simulink model "ADCS_v1"  (R2026a)
settings: Solver=VariableStepAuto  StopTime=t0  FixedStep=0.1  MaxStep=0.1
model workspace (MAT data in the model file):
  i = 8
  omega_thr = 1
  simIn = Simulink.SimulationInput
  simIn.ExternalInput = Simulink.SimulationData.Dataset
  simIn.ExternalInput.any.Name = ''
  simIn.ExternalInput.any.Version = 3
  simIn.ExternalInput.any.Storage = Simulink.SimulationData.Storage.RamDatasetStorage
  simIn.ExternalInput.any.Storage.any.Version = 2
  simIn.ExternalInput.any.Storage.any.Elements{1} = timeseries
  simIn.ExternalInput.any.Storage.any.Elements{1}.Name = 'u1'
  simIn.ExternalInput.any.Storage.any.Elements{1}.DataInfo = tsdata.datametadata
  simIn.ExternalInput.any.Storage.any.Elements{1}.DataInfo.Interpolation = tsdata.interpolation
  simIn.ExternalInput.any.Storage.any.Elements{1}.DataInfo.Interpolation.Fhandle : function handle (value not decoded)
  simIn.ExternalInput.any.Storage.any.Elements{1}.DataInfo.Interpolation.Name = 'linear'
  simIn.ExternalInput.any.Storage.any.Elements{1}.TimeInfo = tsdata.timemetadata
  simIn.ExternalInput.any.Storage.any.Elements{1}.TimeInfo.Length = 101
  simIn.ExternalInput.any.Storage.any.Elements{1}.TimeInfo.DuplicateTimes = 0
  simIn.ExternalInput.any.Storage.any.Elements{1}.TimeInfo.Time_ = [0; 0.1; 0.2; 0.3; 0.4; 0.5; 0.6; 0.7; 0.8; 0.9; 1; 1.1; 1.2; 1.3; 1.4; 1.5; 1.6; 1.7; 1.8; 1.9; 2; 2.1; 2.2; 2.3; 2.4; 2.5; 2.6; 2.7; 2.8; 2.9; 3; 3.1; 3.2; 3.3; 3.4; 3.5; 3.6; 3.7; 3.8; 3.9; 4; 4.1; 4.2; 4.3; 4.4; 4.5; 4.6; 4.7; 4.8; 4.9; 5; 5.1; 5.2; 5.3; 5.4; 5.5; 5.6; 5.7; 5.8; 5.9; 6; 6.1; 6.2; 6.3; 6.4; 6.5; 6.6; 6.7; 6.8; 6.9; 7; 7.1; 7.2; 7.3; 7.4; 7.5; 7.6; 7.7; 7.8; 7.9; 8; 8.1; 8.2; 8.3; 8.4; 8.5; 8.6; 8.7; 8.8; 8.9; 9; 9.1; 9.2; 9.3; 9.4; 9.5; 9.6; 9.7; 9.8; 9.9; 10]
  simIn.ExternalInput.any.Storage.any.Elements{1}.TimeInfo.Initialized = 1
  simIn.ExternalInput.any.Storage.any.Elements{1}.QualityInfo = tsdata.qualmetadata
  simIn.ExternalInput.any.Storage.any.Elements{1}.Data_ = [12; 12; 12; 12; 12; 12; 12; 12; 12; 12; 12; 12; 12; 12; 12; 12; 12; 12; 12; 12; 12; 12; 12; 12; 12; 12; 12; 12; 12; 12; 12; 12; 12; 12; 12; 12; 12; 12; 12; 12; 12; 12; 12; 12; 12; 12; 12; 12; 12; 12; 12; 12; 12; 12; 12; 12; 12; 12; 12; 12; 12; 12; 12; 12; 12; 12; 12; 12; 12; 12; 12; 12; 12; 12; 12; 12; 12; 12; 12; 12; 12; 12; 12; 12; 12; 12; 12; 12; 12; 12; 12; 12; 12; 12; 12; 12; 12; 12; 12; 12; 12]
  simIn.ExternalInput.any.Storage.any.Elements{2} = timeseries
  simIn.ExternalInput.any.Storage.any.Elements{2}.Name = 'u2'
  simIn.ExternalInput.any.Storage.any.Elements{2}.DataInfo = tsdata.datametadata
  simIn.ExternalInput.any.Storage.any.Elements{2}.DataInfo.Interpolation = tsdata.interpolation
  simIn.ExternalInput.any.Storage.any.Elements{2}.DataInfo.Interpolation.Fhandle : function handle (value not decoded)
  simIn.ExternalInput.any.Storage.any.Elements{2}.DataInfo.Interpolation.Name = 'linear'
  simIn.ExternalInput.any.Storage.any.Elements{2}.TimeInfo = tsdata.timemetadata
  simIn.ExternalInput.any.Storage.any.Elements{2}.TimeInfo.Length = 101
  simIn.ExternalInput.any.Storage.any.Elements{2}.TimeInfo.DuplicateTimes = 0
  simIn.ExternalInput.any.Storage.any.Elements{2}.TimeInfo.Time_ = [0; 0.1; 0.2; 0.3; 0.4; 0.5; 0.6; 0.7; 0.8; 0.9; 1; 1.1; 1.2; 1.3; 1.4; 1.5; 1.6; 1.7; 1.8; 1.9; 2; 2.1; 2.2; 2.3; 2.4; 2.5; 2.6; 2.7; 2.8; 2.9; 3; 3.1; 3.2; 3.3; 3.4; 3.5; 3.6; 3.7; 3.8; 3.9; 4; 4.1; 4.2; 4.3; 4.4; 4.5; 4.6; 4.7; 4.8; 4.9; 5; 5.1; 5.2; 5.3; 5.4; 5.5; 5.6; 5.7; 5.8; 5.9; 6; 6.1; 6.2; 6.3; 6.4; 6.5; 6.6; 6.7; 6.8; 6.9; 7; 7.1; 7.2; 7.3; 7.4; 7.5; 7.6; 7.7; 7.8; 7.9; 8; 8.1; 8.2; 8.3; 8.4; 8.5; 8.6; 8.7; 8.8; 8.9; 9; 9.1; 9.2; 9.3; 9.4; 9.5; 9.6; 9.7; 9.8; 9.9; 10]
  simIn.ExternalInput.any.Storage.any.Elements{2}.TimeInfo.Initialized = 1
  simIn.ExternalInput.any.Storage.any.Elements{2}.QualityInfo = tsdata.qualmetadata
  simIn.ExternalInput.any.Storage.any.Elements{2}.Data_ = [1; 1; 1; 1; 1; 1; 1; 1; 1; 1; 1; 1; 1; 1; 1; 1; 1; 1; 1; 1; 1; 1; 1; 1; 1; 1; 1; 1; 1; 1; 1; 1; 1; 1; 1; 1; 1; 1; 1; 1; 1; 1; 1; 1; 1; 1; 1; 1; 1; 1; 1; 1; 1; 1; 1; 1; 1; 1; 1; 1; 1; 1; 1; 1; 1; 1; 1; 1; 1; 1; 1; 1; 1; 1; 1; 1; 1; 1; 1; 1; 1; 1; 1; 1; 1; 1; 1; 1; 1; 1; 1; 1; 1; 1; 1; 1; 1; 1; 1; 1; 1]
  simIn.ExternalInput.any.Storage.any.Elements{3} = timeseries
  simIn.ExternalInput.any.Storage.any.Elements{3}.Name = 'u3'
  simIn.ExternalInput.any.Storage.any.Elements{3}.DataInfo = tsdata.datametadata
  simIn.ExternalInput.any.Storage.any.Elements{3}.DataInfo.Interpolation = tsdata.interpolation
  simIn.ExternalInput.any.Storage.any.Elements{3}.DataInfo.Interpolation.Fhandle : function handle (value not decoded)
  simIn.ExternalInput.any.Storage.any.Elements{3}.DataInfo.Interpolation.Name = 'linear'
  simIn.ExternalInput.any.Storage.any.Elements{3}.TimeInfo = tsdata.timemetadata
  simIn.ExternalInput.any.Storage.any.Elements{3}.TimeInfo.Length = 101
  simIn.ExternalInput.any.Storage.any.Elements{3}.TimeInfo.DuplicateTimes = 0
  simIn.ExternalInput.any.Storage.any.Elements{3}.TimeInfo.Time_ = [0; 0.1; 0.2; 0.3; 0.4; 0.5; 0.6; 0.7; 0.8; 0.9; 1; 1.1; 1.2; 1.3; 1.4; 1.5; 1.6; 1.7; 1.8; 1.9; 2; 2.1; 2.2; 2.3; 2.4; 2.5; 2.6; 2.7; 2.8; 2.9; 3; 3.1; 3.2; 3.3; 3.4; 3.5; 3.6; 3.7; 3.8; 3.9; 4; 4.1; 4.2; 4.3; 4.4; 4.5; 4.6; 4.7; 4.8; 4.9; 5; 5.1; 5.2; 5.3; 5.4; 5.5; 5.6; 5.7; 5.8; 5.9; 6; 6.1; 6.2; 6.3; 6.4; 6.5; 6.6; 6.7; 6.8; 6.9; 7; 7.1; 7.2; 7.3; 7.4; 7.5; 7.6; 7.7; 7.8; 7.9; 8; 8.1; 8.2; 8.3; 8.4; 8.5; 8.6; 8.7; 8.8; 8.9; 9; 9.1; 9.2; 9.3; 9.4; 9.5; 9.6; 9.7; 9.8; 9.9; 10]
  simIn.ExternalInput.any.Storage.any.Elements{3}.TimeInfo.Initialized = 1
  simIn.ExternalInput.any.Storage.any.Elements{3}.QualityInfo = tsdata.qualmetadata
  simIn.ExternalInput.any.Storage.any.Elements{3}.Data_ = [0; 0; 0; 0; 0; 0; 0; 0; 0; 0; 0; 0; 0; 0; 0; 0; 0; 0; 0; 0; 0; 0; 0; 0; 0; 0; 0; 0; 0; 0; 0; 0; 0; 0; 0; 0; 0; 0; 0; 0; 0; 0; 0; 0; 0; 0; 0; 0; 0; 0; 0; 0; 0; 0; 0; 0; 0; 0; 0; 0; 0; 0; 0; 0; 0; 0; 0; 0; 0; 0; 0; 0; 0; 0; 0; 0; 0; 0; 0; 0; 0; 0; 0; 0; 0; 0; 0; 0; 0; 0; 0; 0; 0; 0; 0; 0; 0; 0; 0; 0; 0]
  simIn.ExternalInput.any.Storage.any.Elements{4} = timeseries
  simIn.ExternalInput.any.Storage.any.Elements{4}.Name = 'u4'
  simIn.ExternalInput.any.Storage.any.Elements{4}.DataInfo = tsdata.datametadata
  simIn.ExternalInput.any.Storage.any.Elements{4}.DataInfo.Interpolation = tsdata.interpolation
  simIn.ExternalInput.any.Storage.any.Elements{4}.DataInfo.Interpolation.Fhandle : function handle (value not decoded)
  simIn.ExternalInput.any.Storage.any.Elements{4}.DataInfo.Interpolation.Name = 'linear'
  simIn.ExternalInput.any.Storage.any.Elements{4}.TimeInfo = tsdata.timemetadata
  simIn.ExternalInput.any.Storage.any.Elements{4}.TimeInfo.Length = 101
  simIn.ExternalInput.any.Storage.any.Elements{4}.TimeInfo.DuplicateTimes = 0
  simIn.ExternalInput.any.Storage.any.Elements{4}.TimeInfo.Time_ = [0; 0.1; 0.2; 0.3; 0.4; 0.5; 0.6; 0.7; 0.8; 0.9; 1; 1.1; 1.2; 1.3; 1.4; 1.5; 1.6; 1.7; 1.8; 1.9; 2; 2.1; 2.2; 2.3; 2.4; 2.5; 2.6; 2.7; 2.8; 2.9; 3; 3.1; 3.2; 3.3; 3.4; 3.5; 3.6; 3.7; 3.8; 3.9; 4; 4.1; 4.2; 4.3; 4.4; 4.5; 4.6; 4.7; 4.8; 4.9; 5; 5.1; 5.2; 5.3; 5.4; 5.5; 5.6; 5.7; 5.8; 5.9; 6; 6.1; 6.2; 6.3; 6.4; 6.5; 6.6; 6.7; 6.8; 6.9; 7; 7.1; 7.2; 7.3; 7.4; 7.5; 7.6; 7.7; 7.8; 7.9; 8; 8.1; 8.2; 8.3; 8.4; 8.5; 8.6; 8.7; 8.8; 8.9; 9; 9.1; 9.2; 9.3; 9.4; 9.5; 9.6; 9.7; 9.8; 9.9; 10]
  simIn.ExternalInput.any.Storage.any.Elements{4}.TimeInfo.Initialized = 1
  simIn.ExternalInput.any.Storage.any.Elements{4}.QualityInfo = tsdata.qualmetadata
  simIn.ExternalInput.any.Storage.any.Elements{4}.Data_ = [1; 1; 1; 1; 1; 1; 1; 1; 1; 1; 1; 1; 1; 1; 1; 1; 1; 1; 1; 1; 1; 1; 1; 1; 1; 1; 1; 1; 1; 1; 1; 1; 1; 1; 1; 1; 1; 1; 1; 1; 1; 1; 1; 1; 1; 1; 1; 1; 1; 1; 1; 1; 1; 1; 1; 1; 1; 1; 1; 1; 1; 1; 1; 1; 1; 1; 1; 1; 1; 1; 1; 1; 1; 1; 1; 1; 1; 1; 1; 1; 1; 1; 1; 1; 1; 1; 1; 1; 1; 1; 1; 1; 1; 1; 1; 1; 1; 1; 1; 1; 1]
  simIn.ExternalInput.any.Storage.any.Elements{5} = timeseries
  simIn.ExternalInput.any.Storage.any.Elements{5}.Name = 'u5'
  simIn.ExternalInput.any.Storage.any.Elements{5}.DataInfo = tsdata.datametadata
  simIn.ExternalInput.any.Storage.any.Elements{5}.DataInfo.Interpolation = tsdata.interpolation
  simIn.ExternalInput.any.Storage.any.Elements{5}.DataInfo.Interpolation.Fhandle : function handle (value not decoded)
  simIn.ExternalInput.any.Storage.any.Elements{5}.DataInfo.Interpolation.Name = 'linear'
  simIn.ExternalInput.any.Storage.any.Elements{5}.TimeInfo = tsdata.timemetadata
  simIn.ExternalInput.any.Storage.any.Elements{5}.TimeInfo.Length = 101
  simIn.ExternalInput.any.Storage.any.Elements{5}.TimeInfo.DuplicateTimes = 0
  simIn.ExternalInput.any.Storage.any.Elements{5}.TimeInfo.Time_ = [0; 0.1; 0.2; 0.3; 0.4; 0.5; 0.6; 0.7; 0.8; 0.9; 1; 1.1; 1.2; 1.3; 1.4; 1.5; 1.6; 1.7; 1.8; 1.9; 2; 2.1; 2.2; 2.3; 2.4; 2.5; 2.6; 2.7; 2.8; 2.9; 3; 3.1; 3.2; 3.3; 3.4; 3.5; 3.6; 3.7; 3.8; 3.9; 4; 4.1; 4.2; 4.3; 4.4; 4.5; 4.6; 4.7; 4.8; 4.9; 5; 5.1; 5.2; 5.3; 5.4; 5.5; 5.6; 5.7; 5.8; 5.9; 6; 6.1; 6.2; 6.3; 6.4; 6.5; 6.6; 6.7; 6.8; 6.9; 7; 7.1; 7.2; 7.3; 7.4; 7.5; 7.6; 7.7; 7.8; 7.9; 8; 8.1; 8.2; 8.3; 8.4; 8.5; 8.6; 8.7; 8.8; 8.9; 9; 9.1; 9.2; 9.3; 9.4; 9.5; 9.6; 9.7; 9.8; 9.9; 10]
  simIn.ExternalInput.any.Storage.any.Elements{5}.TimeInfo.Initialized = 1
  simIn.ExternalInput.any.Storage.any.Elements{5}.QualityInfo = tsdata.qualmetadata
  simIn.ExternalInput.any.Storage.any.Elements{5}.Data_ = [0; 0; 0; 0; 0; 0; 0; 0; 0; 0; 0; 0; 0; 0; 0; 0; 0; 0; 0; 0; 0; 0; 0; 0; 0; 0; 0; 0; 0; 0; 0; 0; 0; 0; 0; 0; 0; 0; 0; 0; 0; 0; 0; 0; 0; 0; 0; 0; 0; 0; 0; 0; 0; 0; 0; 0; 0; 0; 0; 0; 0; 0; 0; 0; 0; 0; 0; 0; 0; 0; 0; 0; 0; 0; 0; 0; 0; 0; 0; 0; 0; 0; 0; 0; 0; 0; 0; 0; 0; 0; 0; 0; 0; 0; 0; 0; 0; 0; 0; 0; 0]
  simIn.ExternalInput.any.Storage.any.Elements{6} = timeseries
  simIn.ExternalInput.any.Storage.any.Elements{6}.Name = 'u6'
  simIn.ExternalInput.any.Storage.any.Elements{6}.DataInfo = tsdata.datametadata
  simIn.ExternalInput.any.Storage.any.Elements{6}.DataInfo.Interpolation = tsdata.interpolation
  simIn.ExternalInput.any.Storage.any.Elements{6}.DataInfo.Interpolation.Fhandle : function handle (value not decoded)
  simIn.ExternalInput.any.Storage.any.Elements{6}.DataInfo.Interpolation.Name = 'linear'
  simIn.ExternalInput.any.Storage.any.Elements{6}.TimeInfo = tsdata.timemetadata
  simIn.ExternalInput.any.Storage.any.Elements{6}.TimeInfo.Length = 101
  simIn.ExternalInput.any.Storage.any.Elements{6}.TimeInfo.DuplicateTimes = 0
  simIn.ExternalInput.any.Storage.any.Elements{6}.TimeInfo.Time_ = [0; 0.1; 0.2; 0.3; 0.4; 0.5; 0.6; 0.7; 0.8; 0.9; 1; 1.1; 1.2; 1.3; 1.4; 1.5; 1.6; 1.7; 1.8; 1.9; 2; 2.1; 2.2; 2.3; 2.4; 2.5; 2.6; 2.7; 2.8; 2.9; 3; 3.1; 3.2; 3.3; 3.4; 3.5; 3.6; 3.7; 3.8; 3.9; 4; 4.1; 4.2; 4.3; 4.4; 4.5; 4.6; 4.7; 4.8; 4.9; 5; 5.1; 5.2; 5.3; 5.4; 5.5; 5.6; 5.7; 5.8; 5.9; 6; 6.1; 6.2; 6.3; 6.4; 6.5; 6.6; 6.7; 6.8; 6.9; 7; 7.1; 7.2; 7.3; 7.4; 7.5; 7.6; 7.7; 7.8; 7.9; 8; 8.1; 8.2; 8.3; 8.4; 8.5; 8.6; 8.7; 8.8; 8.9; 9; 9.1; 9.2; 9.3; 9.4; 9.5; 9.6; 9.7; 9.8; 9.9; 10]
  simIn.ExternalInput.any.Storage.any.Elements{6}.TimeInfo.Initialized = 1
  simIn.ExternalInput.any.Storage.any.Elements{6}.QualityInfo = tsdata.qualmetadata
  simIn.ExternalInput.any.Storage.any.Elements{6}.Data_ = [1; 1; 1; 1; 1; 1; 1; 1; 1; 1; 1; 1; 1; 1; 1; 1; 1; 1; 1; 1; 1; 1; 1; 1; 1; 1; 1; 1; 1; 1; 1; 1; 1; 1; 1; 1; 1; 1; 1; 1; 1; 1; 1; 1; 1; 1; 1; 1; 1; 1; 1; 1; 1; 1; 1; 1; 1; 1; 1; 1; 1; 1; 1; 1; 1; 1; 1; 1; 1; 1; 1; 1; 1; 1; 1; 1; 1; 1; 1; 1; 1; 1; 1; 1; 1; 1; 1; 1; 1; 1; 1; 1; 1; 1; 1; 1; 1; 1; 1; 1; 1]
  simIn.ExternalInput.any.Storage.any.Elements{7} = timeseries
  simIn.ExternalInput.any.Storage.any.Elements{7}.Name = 'u7'
  simIn.ExternalInput.any.Storage.any.Elements{7}.DataInfo = tsdata.datametadata
  simIn.ExternalInput.any.Storage.any.Elements{7}.DataInfo.Interpolation = tsdata.interpolation
  simIn.ExternalInput.any.Storage.any.Elements{7}.DataInfo.Interpolation.Fhandle : function handle (value not decoded)
  simIn.ExternalInput.any.Storage.any.Elements{7}.DataInfo.Interpolation.Name = 'linear'
  simIn.ExternalInput.any.Storage.any.Elements{7}.TimeInfo = tsdata.timemetadata
  simIn.ExternalInput.any.Storage.any.Elements{7}.TimeInfo.Length = 101
  simIn.ExternalInput.any.Storage.any.Elements{7}.TimeInfo.DuplicateTimes = 0
  simIn.ExternalInput.any.Storage.any.Elements{7}.TimeInfo.Time_ = [0; 0.1; 0.2; 0.3; 0.4; 0.5; 0.6; 0.7; 0.8; 0.9; 1; 1.1; 1.2; 1.3; 1.4; 1.5; 1.6; 1.7; 1.8; 1.9; 2; 2.1; 2.2; 2.3; 2.4; 2.5; 2.6; 2.7; 2.8; 2.9; 3; 3.1; 3.2; 3.3; 3.4; 3.5; 3.6; 3.7; 3.8; 3.9; 4; 4.1; 4.2; 4.3; 4.4; 4.5; 4.6; 4.7; 4.8; 4.9; 5; 5.1; 5.2; 5.3; 5.4; 5.5; 5.6; 5.7; 5.8; 5.9; 6; 6.1; 6.2; 6.3; 6.4; 6.5; 6.6; 6.7; 6.8; 6.9; 7; 7.1; 7.2; 7.3; 7.4; 7.5; 7.6; 7.7; 7.8; 7.9; 8; 8.1; 8.2; 8.3; 8.4; 8.5; 8.6; 8.7; 8.8; 8.9; 9; 9.1; 9.2; 9.3; 9.4; 9.5; 9.6; 9.7; 9.8; 9.9; 10]
  simIn.ExternalInput.any.Storage.any.Elements{7}.TimeInfo.Initialized = 1
  simIn.ExternalInput.any.Storage.any.Elements{7}.QualityInfo = tsdata.qualmetadata
  simIn.ExternalInput.any.Storage.any.Elements{7}.Data_ = [1; 1; 1; 1; 1; 1; 1; 1; 1; 1; 1; 1; 1; 1; 1; 1; 1; 1; 1; 1; 1; 1; 1; 1; 1; 1; 1; 1; 1; 1; 1; 1; 1; 1; 1; 1; 1; 1; 1; 1; 1; 1; 1; 1; 1; 1; 1; 1; 1; 1; 1; 1; 1; 1; 1; 1; 1; 1; 1; 1; 1; 1; 1; 1; 1; 1; 1; 1; 1; 1; 1; 1; 1; 1; 1; 1; 1; 1; 1; 1; 1; 1; 1; 1; 1; 1; 1; 1; 1; 1; 1; 1; 1; 1; 1; 1; 1; 1; 1; 1; 1]
  simIn.ExternalInput.any.Storage.any.Elements{8} = timeseries
  simIn.ExternalInput.any.Storage.any.Elements{8}.Name = 'u8'
  simIn.ExternalInput.any.Storage.any.Elements{8}.DataInfo = tsdata.datametadata
  simIn.ExternalInput.any.Storage.any.Elements{8}.DataInfo.Interpolation = tsdata.interpolation
  simIn.ExternalInput.any.Storage.any.Elements{8}.DataInfo.Interpolation.Fhandle : function handle (value not decoded)
  simIn.ExternalInput.any.Storage.any.Elements{8}.DataInfo.Interpolation.Name = 'linear'
  simIn.ExternalInput.any.Storage.any.Elements{8}.TimeInfo = tsdata.timemetadata
  simIn.ExternalInput.any.Storage.any.Elements{8}.TimeInfo.Length = 101
  simIn.ExternalInput.any.Storage.any.Elements{8}.TimeInfo.DuplicateTimes = 0
  simIn.ExternalInput.any.Storage.any.Elements{8}.TimeInfo.Time_ = [0; 0.1; 0.2; 0.3; 0.4; 0.5; 0.6; 0.7; 0.8; 0.9; 1; 1.1; 1.2; 1.3; 1.4; 1.5; 1.6; 1.7; 1.8; 1.9; 2; 2.1; 2.2; 2.3; 2.4; 2.5; 2.6; 2.7; 2.8; 2.9; 3; 3.1; 3.2; 3.3; 3.4; 3.5; 3.6; 3.7; 3.8; 3.9; 4; 4.1; 4.2; 4.3; 4.4; 4.5; 4.6; 4.7; 4.8; 4.9; 5; 5.1; 5.2; 5.3; 5.4; 5.5; 5.6; 5.7; 5.8; 5.9; 6; 6.1; 6.2; 6.3; 6.4; 6.5; 6.6; 6.7; 6.8; 6.9; 7; 7.1; 7.2; 7.3; 7.4; 7.5; 7.6; 7.7; 7.8; 7.9; 8; 8.1; 8.2; 8.3; 8.4; 8.5; 8.6; 8.7; 8.8; 8.9; 9; 9.1; 9.2; 9.3; 9.4; 9.5; 9.6; 9.7; 9.8; 9.9; 10]
  simIn.ExternalInput.any.Storage.any.Elements{8}.TimeInfo.Initialized = 1
  simIn.ExternalInput.any.Storage.any.Elements{8}.QualityInfo = tsdata.qualmetadata
  simIn.ExternalInput.any.Storage.any.Elements{8}.Data_ = [0; 0; 0; 0; 0; 0; 0; 0; 0; 0; 0; 0; 0; 0; 0; 0; 0; 0; 0; 0; 0; 0; 0; 0; 0; 0; 0; 0; 0; 0; 0; 0; 0; 0; 0; 0; 0; 0; 0; 0; 0; 0; 0; 0; 0; 0; 0; 0; 0; 0; 0; 0; 0; 0; 0; 0; 0; 0; 0; 0; 0; 0; 0; 0; 0; 0; 0; 0; 0; 0; 0; 0; 0; 0; 0; 0; 0; 0; 0; 0; 0; 0; 0; 0; 0; 0; 0; 0; 0; 0; 0; 0; 0; 0; 0; 0; 0; 0; 0; 0; 0]
  simIn.ExternalInput.any.Storage.any.Elements{9} = timeseries
  simIn.ExternalInput.any.Storage.any.Elements{9}.Name = 'u9'
  simIn.ExternalInput.any.Storage.any.Elements{9}.DataInfo = tsdata.datametadata
  simIn.ExternalInput.any.Storage.any.Elements{9}.DataInfo.Interpolation = tsdata.interpolation
  simIn.ExternalInput.any.Storage.any.Elements{9}.DataInfo.Interpolation.Fhandle : function handle (value not decoded)
  simIn.ExternalInput.any.Storage.any.Elements{9}.DataInfo.Interpolation.Name = 'linear'
  simIn.ExternalInput.any.Storage.any.Elements{9}.TimeInfo = tsdata.timemetadata
  simIn.ExternalInput.any.Storage.any.Elements{9}.TimeInfo.Length = 101
  simIn.ExternalInput.any.Storage.any.Elements{9}.TimeInfo.DuplicateTimes = 0
  simIn.ExternalInput.any.Storage.any.Elements{9}.TimeInfo.Time_ = [0; 0.1; 0.2; 0.3; 0.4; 0.5; 0.6; 0.7; 0.8; 0.9; 1; 1.1; 1.2; 1.3; 1.4; 1.5; 1.6; 1.7; 1.8; 1.9; 2; 2.1; 2.2; 2.3; 2.4; 2.5; 2.6; 2.7; 2.8; 2.9; 3; 3.1; 3.2; 3.3; 3.4; 3.5; 3.6; 3.7; 3.8; 3.9; 4; 4.1; 4.2; 4.3; 4.4; 4.5; 4.6; 4.7; 4.8; 4.9; 5; 5.1; 5.2; 5.3; 5.4; 5.5; 5.6; 5.7; 5.8; 5.9; 6; 6.1; 6.2; 6.3; 6.4; 6.5; 6.6; 6.7; 6.8; 6.9; 7; 7.1; 7.2; 7.3; 7.4; 7.5; 7.6; 7.7; 7.8; 7.9; 8; 8.1; 8.2; 8.3; 8.4; 8.5; 8.6; 8.7; 8.8; 8.9; 9; 9.1; 9.2; 9.3; 9.4; 9.5; 9.6; 9.7; 9.8; 9.9; 10]
  simIn.ExternalInput.any.Storage.any.Elements{9}.TimeInfo.Initialized = 1
  simIn.ExternalInput.any.Storage.any.Elements{9}.QualityInfo = tsdata.qualmetadata
  simIn.ExternalInput.any.Storage.any.Elements{9}.Data_ = [1; 1; 1; 1; 1; 1; 1; 1; 1; 1; 1; 1; 1; 1; 1; 1; 1; 1; 1; 1; 1; 1; 1; 1; 1; 1; 1; 1; 1; 1; 1; 1; 1; 1; 1; 1; 1; 1; 1; 1; 1; 1; 1; 1; 1; 1; 1; 1; 1; 1; 1; 1; 1; 1; 1; 1; 1; 1; 1; 1; 1; 1; 1; 1; 1; 1; 1; 1; 1; 1; 1; 1; 1; 1; 1; 1; 1; 1; 1; 1; 1; 1; 1; 1; 1; 1; 1; 1; 1; 1; 1; 1; 1; 1; 1; 1; 1; 1; 1; 1; 1]
  simIn.ExternalInput.any.Storage.any.Elements{10} = timeseries
  simIn.ExternalInput.any.Storage.any.Elements{10}.Name = 'u10'
  simIn.ExternalInput.any.Storage.any.Elements{10}.DataInfo = tsdata.datametadata
  simIn.ExternalInput.any.Storage.any.Elements{10}.DataInfo.Interpolation = tsdata.interpolation
  simIn.ExternalInput.any.Storage.any.Elements{10}.DataInfo.Interpolation.Fhandle : function handle (value not decoded)
  simIn.ExternalInput.any.Storage.any.Elements{10}.DataInfo.Interpolation.Name = 'linear'
  simIn.ExternalInput.any.Storage.any.Elements{10}.TimeInfo = tsdata.timemetadata
  simIn.ExternalInput.any.Storage.any.Elements{10}.TimeInfo.Length = 101
  simIn.ExternalInput.any.Storage.any.Elements{10}.TimeInfo.DuplicateTimes = 0
  simIn.ExternalInput.any.Storage.any.Elements{10}.TimeInfo.Time_ = [0; 0.1; 0.2; 0.3; 0.4; 0.5; 0.6; 0.7; 0.8; 0.9; 1; 1.1; 1.2; 1.3; 1.4; 1.5; 1.6; 1.7; 1.8; 1.9; 2; 2.1; 2.2; 2.3; 2.4; 2.5; 2.6; 2.7; 2.8; 2.9; 3; 3.1; 3.2; 3.3; 3.4; 3.5; 3.6; 3.7; 3.8; 3.9; 4; 4.1; 4.2; 4.3; 4.4; 4.5; 4.6; 4.7; 4.8; 4.9; 5; 5.1; 5.2; 5.3; 5.4; 5.5; 5.6; 5.7; 5.8; 5.9; 6; 6.1; 6.2; 6.3; 6.4; 6.5; 6.6; 6.7; 6.8; 6.9; 7; 7.1; 7.2; 7.3; 7.4; 7.5; 7.6; 7.7; 7.8; 7.9; 8; 8.1; 8.2; 8.3; 8.4; 8.5; 8.6; 8.7; 8.8; 8.9; 9; 9.1; 9.2; 9.3; 9.4; 9.5; 9.6; 9.7; 9.8; 9.9; 10]
  simIn.ExternalInput.any.Storage.any.Elements{10}.TimeInfo.Initialized = 1
  simIn.ExternalInput.any.Storage.any.Elements{10}.QualityInfo = tsdata.qualmetadata
  simIn.ExternalInput.any.Storage.any.Elements{10}.Data_ = [0; 0; 0; 0; 0; 0; 0; 0; 0; 0; 0; 0; 0; 0; 0; 0; 0; 0; 0; 0; 0; 0; 0; 0; 0; 0; 0; 0; 0; 0; 0; 0; 0; 0; 0; 0; 0; 0; 0; 0; 0; 0; 0; 0; 0; 0; 0; 0; 0; 0; 0; 0; 0; 0; 0; 0; 0; 0; 0; 0; 0; 0; 0; 0; 0; 0; 0; 0; 0; 0; 0; 0; 0; 0; 0; 0; 0; 0; 0; 0; 0; 0; 0; 0; 0; 0; 0; 0; 0; 0; 0; 0; 0; 0; 0; 0; 0; 0; 0; 0; 0]
  simIn.ExternalInput.any.Storage.any.Elements{11} = timeseries
  simIn.ExternalInput.any.Storage.any.Elements{11}.Name = 'u11'
  simIn.ExternalInput.any.Storage.any.Elements{11}.DataInfo = tsdata.datametadata
  simIn.ExternalInput.any.Storage.any.Elements{11}.DataInfo.Interpolation = tsdata.interpolation
  simIn.ExternalInput.any.Storage.any.Elements{11}.DataInfo.Interpolation.Fhandle : function handle (value not decoded)
  simIn.ExternalInput.any.Storage.any.Elements{11}.DataInfo.Interpolation.Name = 'linear'
  simIn.ExternalInput.any.Storage.any.Elements{11}.TimeInfo = tsdata.timemetadata
  simIn.ExternalInput.any.Storage.any.Elements{11}.TimeInfo.Length = 101
  simIn.ExternalInput.any.Storage.any.Elements{11}.TimeInfo.DuplicateTimes = 0
  simIn.ExternalInput.any.Storage.any.Elements{11}.TimeInfo.Time_ = [0; 0.1; 0.2; 0.3; 0.4; 0.5; 0.6; 0.7; 0.8; 0.9; 1; 1.1; 1.2; 1.3; 1.4; 1.5; 1.6; 1.7; 1.8; 1.9; 2; 2.1; 2.2; 2.3; 2.4; 2.5; 2.6; 2.7; 2.8; 2.9; 3; 3.1; 3.2; 3.3; 3.4; 3.5; 3.6; 3.7; 3.8; 3.9; 4; 4.1; 4.2; 4.3; 4.4; 4.5; 4.6; 4.7; 4.8; 4.9; 5; 5.1; 5.2; 5.3; 5.4; 5.5; 5.6; 5.7; 5.8; 5.9; 6; 6.1; 6.2; 6.3; 6.4; 6.5; 6.6; 6.7; 6.8; 6.9; 7; 7.1; 7.2; 7.3; 7.4; 7.5; 7.6; 7.7; 7.8; 7.9; 8; 8.1; 8.2; 8.3; 8.4; 8.5; 8.6; 8.7; 8.8; 8.9; 9; 9.1; 9.2; 9.3; 9.4; 9.5; 9.6; 9.7; 9.8; 9.9; 10]
  simIn.ExternalInput.any.Storage.any.Elements{11}.TimeInfo.Initialized = 1
  simIn.ExternalInput.any.Storage.any.Elements{11}.QualityInfo = tsdata.qualmetadata
  simIn.ExternalInput.any.Storage.any.Elements{11}.Data_ = [1; 1; 1; 1; 1; 1; 1; 1; 1; 1; 1; 1; 1; 1; 1; 1; 1; 1; 1; 1; 1; 1; 1; 1; 1; 1; 1; 1; 1; 1; 1; 1; 1; 1; 1; 1; 1; 1; 1; 1; 1; 1; 1; 1; 1; 1; 1; 1; 1; 1; 1; 1; 1; 1; 1; 1; 1; 1; 1; 1; 1; 1; 1; 1; 1; 1; 1; 1; 1; 1; 1; 1; 1; 1; 1; 1; 1; 1; 1; 1; 1; 1; 1; 1; 1; 1; 1; 1; 1; 1; 1; 1; 1; 1; 1; 1; 1; 1; 1; 1; 1]
  simIn.ExternalInput.any.Storage.any.Elements{12} = timeseries
  simIn.ExternalInput.any.Storage.any.Elements{12}.Name = 'u12'
  simIn.ExternalInput.any.Storage.any.Elements{12}.DataInfo = tsdata.datametadata
  simIn.ExternalInput.any.Storage.any.Elements{12}.DataInfo.Interpolation = tsdata.interpolation
  simIn.ExternalInput.any.Storage.any.Elements{12}.DataInfo.Interpolation.Fhandle : function handle (value not decoded)
  simIn.ExternalInput.any.Storage.any.Elements{12}.DataInfo.Interpolation.Name = 'linear'
  simIn.ExternalInput.any.Storage.any.Elements{12}.TimeInfo = tsdata.timemetadata
  simIn.ExternalInput.any.Storage.any.Elements{12}.TimeInfo.Length = 101
  simIn.ExternalInput.any.Storage.any.Elements{12}.TimeInfo.DuplicateTimes = 0
  simIn.ExternalInput.any.Storage.any.Elements{12}.TimeInfo.Time_ = [0; 0.1; 0.2; 0.3; 0.4; 0.5; 0.6; 0.7; 0.8; 0.9; 1; 1.1; 1.2; 1.3; 1.4; 1.5; 1.6; 1.7; 1.8; 1.9; 2; 2.1; 2.2; 2.3; 2.4; 2.5; 2.6; 2.7; 2.8; 2.9; 3; 3.1; 3.2; 3.3; 3.4; 3.5; 3.6; 3.7; 3.8; 3.9; 4; 4.1; 4.2; 4.3; 4.4; 4.5; 4.6; 4.7; 4.8; 4.9; 5; 5.1; 5.2; 5.3; 5.4; 5.5; 5.6; 5.7; 5.8; 5.9; 6; 6.1; 6.2; 6.3; 6.4; 6.5; 6.6; 6.7; 6.8; 6.9; 7; 7.1; 7.2; 7.3; 7.4; 7.5; 7.6; 7.7; 7.8; 7.9; 8; 8.1; 8.2; 8.3; 8.4; 8.5; 8.6; 8.7; 8.8; 8.9; 9; 9.1; 9.2; 9.3; 9.4; 9.5; 9.6; 9.7; 9.8; 9.9; 10]
  simIn.ExternalInput.any.Storage.any.Elements{12}.TimeInfo.Initialized = 1
  simIn.ExternalInput.any.Storage.any.Elements{12}.QualityInfo = tsdata.qualmetadata
  simIn.ExternalInput.any.Storage.any.Elements{12}.Data_ = [1; 1; 1; 1; 1; 1; 1; 1; 1; 1; 1; 1; 1; 1; 1; 1; 1; 1; 1; 1; 1; 1; 1; 1; 1; 1; 1; 1; 1; 1; 1; 1; 1; 1; 1; 1; 1; 1; 1; 1; 1; 1; 1; 1; 1; 1; 1; 1; 1; 1; 1; 1; 1; 1; 1; 1; 1; 1; 1; 1; 1; 1; 1; 1; 1; 1; 1; 1; 1; 1; 1; 1; 1; 1; 1; 1; 1; 1; 1; 1; 1; 1; 1; 1; 1; 1; 1; 1; 1; 1; 1; 1; 1; 1; 1; 1; 1; 1; 1; 1; 1]
  simIn.ExternalInput.any.Storage.any.Elements{13} = timeseries
  simIn.ExternalInput.any.Storage.any.Elements{13}.Name = 'u13'
  simIn.ExternalInput.any.Storage.any.Elements{13}.DataInfo = tsdata.datametadata
  simIn.ExternalInput.any.Storage.any.Elements{13}.DataInfo.Interpolation = tsdata.interpolation
  simIn.ExternalInput.any.Storage.any.Elements{13}.DataInfo.Interpolation.Fhandle : function handle (value not decoded)
  simIn.ExternalInput.any.Storage.any.Elements{13}.DataInfo.Interpolation.Name = 'linear'
  simIn.ExternalInput.any.Storage.any.Elements{13}.TimeInfo = tsdata.timemetadata
  simIn.ExternalInput.any.Storage.any.Elements{13}.TimeInfo.Length = 101
  simIn.ExternalInput.any.Storage.any.Elements{13}.TimeInfo.DuplicateTimes = 0
  simIn.ExternalInput.any.Storage.any.Elements{13}.TimeInfo.Time_ = [0; 0.1; 0.2; 0.3; 0.4; 0.5; 0.6; 0.7; 0.8; 0.9; 1; 1.1; 1.2; 1.3; 1.4; 1.5; 1.6; 1.7; 1.8; 1.9; 2; 2.1; 2.2; 2.3; 2.4; 2.5; 2.6; 2.7; 2.8; 2.9; 3; 3.1; 3.2; 3.3; 3.4; 3.5; 3.6; 3.7; 3.8; 3.9; 4; 4.1; 4.2; 4.3; 4.4; 4.5; 4.6; 4.7; 4.8; 4.9; 5; 5.1; 5.2; 5.3; 5.4; 5.5; 5.6; 5.7; 5.8; 5.9; 6; 6.1; 6.2; 6.3; 6.4; 6.5; 6.6; 6.7; 6.8; 6.9; 7; 7.1; 7.2; 7.3; 7.4; 7.5; 7.6; 7.7; 7.8; 7.9; 8; 8.1; 8.2; 8.3; 8.4; 8.5; 8.6; 8.7; 8.8; 8.9; 9; 9.1; 9.2; 9.3; 9.4; 9.5; 9.6; 9.7; 9.8; 9.9; 10]
  simIn.ExternalInput.any.Storage.any.Elements{13}.TimeInfo.Initialized = 1
  simIn.ExternalInput.any.Storage.any.Elements{13}.QualityInfo = tsdata.qualmetadata
  simIn.ExternalInput.any.Storage.any.Elements{13}.Data_ = [1; 1; 1; 1; 1; 1; 1; 1; 1; 1; 1; 1; 1; 1; 1; 1; 1; 1; 1; 1; 1; 1; 1; 1; 1; 1; 1; 1; 1; 1; 1; 1; 1; 1; 1; 1; 1; 1; 1; 1; 1; 1; 1; 1; 1; 1; 1; 1; 1; 1; 1; 1; 1; 1; 1; 1; 1; 1; 1; 1; 1; 1; 1; 1; 1; 1; 1; 1; 1; 1; 1; 1; 1; 1; 1; 1; 1; 1; 1; 1; 1; 1; 1; 1; 1; 1; 1; 1; 1; 1; 1; 1; 1; 1; 1; 1; 1; 1; 1; 1; 1]
  simIn.ExternalInput.any.Storage.any.Elements{14} = timeseries
  simIn.ExternalInput.any.Storage.any.Elements{14}.Name = 'u14'
  simIn.ExternalInput.any.Storage.any.Elements{14}.DataInfo = tsdata.datametadata
  simIn.ExternalInput.any.Storage.any.Elements{14}.DataInfo.Interpolation = tsdata.interpolation
  simIn.ExternalInput.any.Storage.any.Elements{14}.DataInfo.Interpolation.Fhandle : function handle (value not decoded)
  simIn.ExternalInput.any.Storage.any.Elements{14}.DataInfo.Interpolation.Name = 'linear'
  simIn.ExternalInput.any.Storage.any.Elements{14}.TimeInfo = tsdata.timemetadata
  simIn.ExternalInput.any.Storage.any.Elements{14}.TimeInfo.Length = 101
  simIn.ExternalInput.any.Storage.any.Elements{14}.TimeInfo.DuplicateTimes = 0
  simIn.ExternalInput.any.Storage.any.Elements{14}.TimeInfo.Time_ = [0; 0.1; 0.2; 0.3; 0.4; 0.5; 0.6; 0.7; 0.8; 0.9; 1; 1.1; 1.2; 1.3; 1.4; 1.5; 1.6; 1.7; 1.8; 1.9; 2; 2.1; 2.2; 2.3; 2.4; 2.5; 2.6; 2.7; 2.8; 2.9; 3; 3.1; 3.2; 3.3; 3.4; 3.5; 3.6; 3.7; 3.8; 3.9; 4; 4.1; 4.2; 4.3; 4.4; 4.5; 4.6; 4.7; 4.8; 4.9; 5; 5.1; 5.2; 5.3; 5.4; 5.5; 5.6; 5.7; 5.8; 5.9; 6; 6.1; 6.2; 6.3; 6.4; 6.5; 6.6; 6.7; 6.8; 6.9; 7; 7.1; 7.2; 7.3; 7.4; 7.5; 7.6; 7.7; 7.8; 7.9; 8; 8.1; 8.2; 8.3; 8.4; 8.5; 8.6; 8.7; 8.8; 8.9; 9; 9.1; 9.2; 9.3; 9.4; 9.5; 9.6; 9.7; 9.8; 9.9; 10]
  simIn.ExternalInput.any.Storage.any.Elements{14}.TimeInfo.Initialized = 1
  simIn.ExternalInput.any.Storage.any.Elements{14}.QualityInfo = tsdata.qualmetadata
  simIn.ExternalInput.any.Storage.any.Elements{14}.Data_ = [1; 1; 1; 1; 1; 1; 1; 1; 1; 1; 1; 1; 1; 1; 1; 1; 1; 1; 1; 1; 1; 1; 1; 1; 1; 1; 1; 1; 1; 1; 1; 1; 1; 1; 1; 1; 1; 1; 1; 1; 1; 1; 1; 1; 1; 1; 1; 1; 1; 1; 1; 1; 1; 1; 1; 1; 1; 1; 1; 1; 1; 1; 1; 1; 1; 1; 1; 1; 1; 1; 1; 1; 1; 1; 1; 1; 1; 1; 1; 1; 1; 1; 1; 1; 1; 1; 1; 1; 1; 1; 1; 1; 1; 1; 1; 1; 1; 1; 1; 1; 1]
  simIn.ExternalInput.any.Storage.any.Elements{15} = timeseries
  simIn.ExternalInput.any.Storage.any.Elements{15}.Name = 'u15'
  simIn.ExternalInput.any.Storage.any.Elements{15}.DataInfo = tsdata.datametadata
  simIn.ExternalInput.any.Storage.any.Elements{15}.DataInfo.Interpolation = tsdata.interpolation
  simIn.ExternalInput.any.Storage.any.Elements{15}.DataInfo.Interpolation.Fhandle : function handle (value not decoded)
  simIn.ExternalInput.any.Storage.any.Elements{15}.DataInfo.Interpolation.Name = 'linear'
  simIn.ExternalInput.any.Storage.any.Elements{15}.TimeInfo = tsdata.timemetadata
  simIn.ExternalInput.any.Storage.any.Elements{15}.TimeInfo.Length = 101
  simIn.ExternalInput.any.Storage.any.Elements{15}.TimeInfo.DuplicateTimes = 0
  simIn.ExternalInput.any.Storage.any.Elements{15}.TimeInfo.Time_ = [0; 0.1; 0.2; 0.3; 0.4; 0.5; 0.6; 0.7; 0.8; 0.9; 1; 1.1; 1.2; 1.3; 1.4; 1.5; 1.6; 1.7; 1.8; 1.9; 2; 2.1; 2.2; 2.3; 2.4; 2.5; 2.6; 2.7; 2.8; 2.9; 3; 3.1; 3.2; 3.3; 3.4; 3.5; 3.6; 3.7; 3.8; 3.9; 4; 4.1; 4.2; 4.3; 4.4; 4.5; 4.6; 4.7; 4.8; 4.9; 5; 5.1; 5.2; 5.3; 5.4; 5.5; 5.6; 5.7; 5.8; 5.9; 6; 6.1; 6.2; 6.3; 6.4; 6.5; 6.6; 6.7; 6.8; 6.9; 7; 7.1; 7.2; 7.3; 7.4; 7.5; 7.6; 7.7; 7.8; 7.9; 8; 8.1; 8.2; 8.3; 8.4; 8.5; 8.6; 8.7; 8.8; 8.9; 9; 9.1; 9.2; 9.3; 9.4; 9.5; 9.6; 9.7; 9.8; 9.9; 10]
  simIn.ExternalInput.any.Storage.any.Elements{15}.TimeInfo.Initialized = 1
  simIn.ExternalInput.any.Storage.any.Elements{15}.QualityInfo = tsdata.qualmetadata
  simIn.ExternalInput.any.Storage.any.Elements{15}.Data_ = [1; 1; 1; 1; 1; 1; 1; 1; 1; 1; 1; 1; 1; 1; 1; 1; 1; 1; 1; 1; 1; 1; 1; 1; 1; 1; 1; 1; 1; 1; 1; 1; 1; 1; 1; 1; 1; 1; 1; 1; 1; 1; 1; 1; 1; 1; 1; 1; 1; 1; 1; 1; 1; 1; 1; 1; 1; 1; 1; 1; 1; 1; 1; 1; 1; 1; 1; 1; 1; 1; 1; 1; 1; 1; 1; 1; 1; 1; 1; 1; 1; 1; 1; 1; 1; 1; 1; 1; 1; 1; 1; 1; 1; 1; 1; 1; 1; 1; 1; 1; 1]
  simIn.ExternalInput.any.Storage.any.Elements{16} = timeseries
  simIn.ExternalInput.any.Storage.any.Elements{16}.Name = 'u16'
  simIn.ExternalInput.any.Storage.any.Elements{16}.DataInfo = tsdata.datametadata
  simIn.ExternalInput.any.Storage.any.Elements{16}.DataInfo.Interpolation = tsdata.interpolation
  simIn.ExternalInput.any.Storage.any.Elements{16}.DataInfo.Interpolation.Fhandle : function handle (value not decoded)
  simIn.ExternalInput.any.Storage.any.Elements{16}.DataInfo.Interpolation.Name = 'linear'
  simIn.ExternalInput.any.Storage.any.Elements{16}.TimeInfo = tsdata.timemetadata
  simIn.ExternalInput.any.Storage.any.Elements{16}.TimeInfo.Length = 101
  simIn.ExternalInput.any.Storage.any.Elements{16}.TimeInfo.DuplicateTimes = 0
  simIn.ExternalInput.any.Storage.any.Elements{16}.TimeInfo.Time_ = [0; 0.1; 0.2; 0.3; 0.4; 0.5; 0.6; 0.7; 0.8; 0.9; 1; 1.1; 1.2; 1.3; 1.4; 1.5; 1.6; 1.7; 1.8; 1.9; 2; 2.1; 2.2; 2.3; 2.4; 2.5; 2.6; 2.7; 2.8; 2.9; 3; 3.1; 3.2; 3.3; 3.4; 3.5; 3.6; 3.7; 3.8; 3.9; 4; 4.1; 4.2; 4.3; 4.4; 4.5; 4.6; 4.7; 4.8; 4.9; 5; 5.1; 5.2; 5.3; 5.4; 5.5; 5.6; 5.7; 5.8; 5.9; 6; 6.1; 6.2; 6.3; 6.4; 6.5; 6.6; 6.7; 6.8; 6.9; 7; 7.1; 7.2; 7.3; 7.4; 7.5; 7.6; 7.7; 7.8; 7.9; 8; 8.1; 8.2; 8.3; 8.4; 8.5; 8.6; 8.7; 8.8; 8.9; 9; 9.1; 9.2; 9.3; 9.4; 9.5; 9.6; 9.7; 9.8; 9.9; 10]
  simIn.ExternalInput.any.Storage.any.Elements{16}.TimeInfo.Initialized = 1
  simIn.ExternalInput.any.Storage.any.Elements{16}.QualityInfo = tsdata.qualmetadata
  simIn.ExternalInput.any.Storage.any.Elements{16}.Data_ = [0; 0; 0; 0; 0; 0; 0; 0; 0; 0; 0; 0; 0; 0; 0; 0; 0; 0; 0; 0; 0; 0; 0; 0; 0; 0; 0; 0; 0; 0; 0; 0; 0; 0; 0; 0; 0; 0; 0; 0; 0; 0; 0; 0; 0; 0; 0; 0; 0; 0; 0; 0; 0; 0; 0; 0; 0; 0; 0; 0; 0; 0; 0; 0; 0; 0; 0; 0; 0; 0; 0; 0; 0; 0; 0; 0; 0; 0; 0; 0; 0; 0; 0; 0; 0; 0; 0; 0; 0; 0; 0; 0; 0; 0; 0; 0; 0; 0; 0; 0; 0]
  simIn.ExperimentalProperties = Simulink.Simulation.internal.ExperimentalProperties
  simIn.ModelName_ = 'ADCS_FSM_test'
  t = [0; 0.1; 0.2; 0.3; 0.4; 0.5; 0.6; 0.7; 0.8; 0.9; 1; 1.1; 1.2; 1.3; 1.4; 1.5; 1.6; 1.7; 1.8; 1.9; 2; 2.1; 2.2; 2.3; 2.4; 2.5; 2.6; 2.7; 2.8; 2.9; 3; 3.1; 3.2; 3.3; 3.4; 3.5; 3.6; 3.7; 3.8; 3.9; 4; 4.1; 4.2; 4.3; 4.4; 4.5; 4.6; 4.7; 4.8; 4.9; 5; 5.1; 5.2; 5.3; 5.4; 5.5; 5.6; 5.7; 5.8; 5.9; 6; 6.1; 6.2; 6.3; 6.4; 6.5; 6.6; 6.7; 6.8; 6.9; 7; 7.1; 7.2; 7.3; 7.4; 7.5; 7.6; 7.7; 7.8; 7.9; 8; 8.1; 8.2; 8.3; 8.4; 8.5; 8.6; 8.7; 8.8; 8.9; 9; 9.1; 9.2; 9.3; 9.4; 9.5; 9.6; 9.7; 9.8; 9.9; 10]
  u : object (value not decoded)
  y_out = [0 0 0 0 0 0 0 0]
values from neighbouring files (symbols this model uses):
  B = [1 0 0]    [parameters.m]
  h_max = 1.47    [parameters.m]
  I_RW = 1    [parameters.m]
  k_desat = 1    [parameters.m]
  kd_detumble = 1    [parameters.m]
  kd_hold = 1    [parameters.m]
  kd_point = 20    [parameters.m]
  kd_slew_fast = 1    [parameters.m]
  kd_slew_slow = 1    [parameters.m]
  kd_spin = 0    [parameters.m]
  kp_hold = 1    [parameters.m]
  kp_point = 2    [parameters.m]
  kp_slew_fast = 1    [parameters.m]
  kp_slew_slow = 1    [parameters.m]
  kp_spin = 1    [parameters.m]
  omega_0 = [0 0 0.0011]    [parameters.m]
  omega_ref = [0 0 0]    [parameters.m]
  omega_zero = 0.001    [parameters.m]
  P = satellite_params()    [individual_test_with_dynamics.m]    (also in parameters.m; test.m = thrusters(:, 1:3))
  q0 = [sqrt(0.5) -sqrt(0.5) 0 0]    [parameters.m]
  q_ref = [ cos(theta_ref/2) ... (first row only)    [parameters.m]
libraries: matrix_library x13, simulink x6, aerolibutil x4, sim3dlib x2
(part 1 of 2)
settings Model: Creator=ADMIN  LastModifiedBy=Administrator
settings DataIOCC: ExternalInput=ds  LoadExternalInput=on
settings SimscapeCC: SimscapeNominalValues="[{\"value\":\"1\",\"unit\":\"A\"},{\"value\":\"1\",\"unit\":\"bar\"},{\"value\":\"1\",\"unit\":\"cm^2\"},{\"value\":\"1\",\"unit\":\"cm^3/s\"},{\"value\":\"1\",\"unit\":\"kJ/kg\"},{\"value\":\"1\",\"unit\":\"kW\"},{\"value\":\"1\",\"unit\":\"l\"},{\"value\":\"1\",\"unit\":\"N\"},{\"value\":\"1\",\"unit\":\"N*m\"},{\"value\":\"1\",\"unit\":\"V\"}]"  SimscapeLogType=none  SimscapeLogDataHistory=5000.0

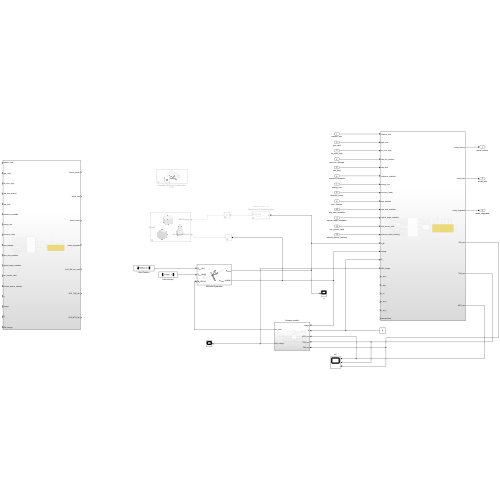
[thumbnail: Simulink's stored preview of the top-level diagram]
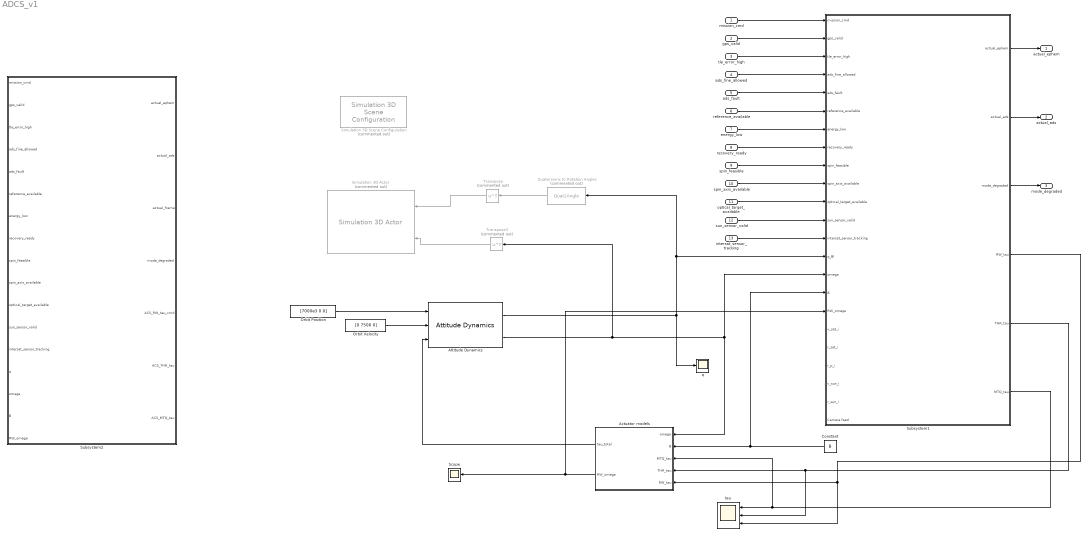
== system ADCS_v1 ==
  mission_cmd : Inport  OutDataTypeStr=uint8  PortDimensions=1
  gps_valid : Inport  Port=2  OutDataTypeStr=boolean  PortDimensions=1
  tle_error_high : Inport  Port=3  OutDataTypeStr=boolean  PortDimensions=1
  ads_fine_allowed : Inport  Port=4  OutDataTypeStr=boolean  PortDimensions=1
  ads_fault : Inport  Port=5  OutDataTypeStr=boolean  PortDimensions=1
  reference_available : Inport  Port=6  OutDataTypeStr=boolean  PortDimensions=1
  energy_low : Inport  Port=7  OutDataTypeStr=boolean  PortDimensions=1
  recovery_ready : Inport  Port=8  OutDataTypeStr=boolean  PortDimensions=1
  spin_feasible : Inport  Port=9  OutDataTypeStr=boolean  PortDimensions=1
  spin_axis_available : Inport  Port=10  OutDataTypeStr=boolean  PortDimensions=1
  optical_target_available : Inport  Port=11  OutDataTypeStr=boolean  PortDimensions=1
  sun_sensor_valid : Inport  Port=12  OutDataTypeStr=boolean  PortDimensions=1
  intersat_sensor_tracking : Inport  Port=13  OutDataTypeStr=boolean  PortDimensions=1
  Actuator models : Subsystem
  Attitude Dynamics : AttitudeDynamics  dateOut=off  mass=P.mass0  inertia=P.I0  outputFuelStatus=off  attitude=q0.'  attitudeRate=omega_0.'  useGravGrad=off  angleUnits=Radians
  Constant : Constant  Value=B
  Orbit Position : Constant  Value=[7000e3 0 0]
  Orbit Velocity : Constant  Value=[0 7500 0]
  Quaternions to Rotation Angles : Quat2Angle  Commented=on
      settings: AttributesFormatString=Rotation Order: %<rotationOrder>
  Scope : Scope
      settings: ActiveDisplayYMinimum=-1  ActiveDisplayYMaximum=1
  Simulation 3D Actor : sim3dlib/Simulation 3D Actor  Priority=1  Commented=on  ActorName=M4V  ParentName=Scene Origin  Operation=Create at setup  InitScriptText=|  SampleTime=-1  Translation=[0 0 0]  Rotation=[0 0 0]  Scale=[1 1 1]*0.1  InputsText="M4V.Rotation        M4V.AngularVelocity"  aMode=5  ActorTag=M4V  ActorType=Sim3dActor  ID=C
      | % Reserved keywords:
      | % - Actor : handle to this actor object
      | % - World : handle to the world object
      | 
      | % Examples:
      | 
      | % Create a primitive geometry (optional)
      | % createShape(Actor, 'box', [1 1 1]);
      | 
      | % Initialize values (optional)
      | % Actor.Physics = true;
      | % Actor.Color = [1 0 0];
      | M4V.Mobility = sim3d.utils.MobilityTypes.Movable;
      | 
      | % For simple motion without gravity
      | M4V.Physics = true;
      | M4V.Gravity = false;
      | M4V.Collisions = false;
  Simulation 3D Scene Configuration : sim3dlib/Simulation 3D Scene Configuration  Priority=0  Commented=on  ProjectFormat=Default Scenes  SceneDesc=Space  ProjectName=C:\Program Files\MATLAB\R2026a\toolbox\shared\sim3d_projects\automotive_project_windows\UE\WindowsNoEditor\VehicleSimulation.exe  ScenePath=/Game/Maps/HwStrght  EnableOpenDRIVE=off  vehTagList={'Custom';'M4V';'Scene Origin';'sun'}  vehTag=Custom  AttachedCameraRelativeTranslation=[-20000 0 0]  FreeCameraDefaultInitialTranslation=[-6, 0, 2]  AttachedCameraRelativeRotation=[0 0 0]  FreeCameraDefaultInitialRotation=[0, -15, 0]  ViewpointName=Custom  FreeCameraInitialTranslation=[-1500 0 500]  FreeCameraInitialRotation=[0 0 0]  OpVisEn=off  Ts=1  EnableWindow=on  EnableRemoteAccess=off  SimulationMode=CoSimulation  SimulateUsing=Interpreted execution  EnableAnimationRecording=off  OverrideDefaultRecording=off  AnimationRecordingFileName=sim3dAnimation.mat  AnimationRecordingInterval=[0 inf]  EnableWeather=off  SunAzimuth=90  SunAltitude=40.0  EnableGeospatialSun=off  Latitude=0  Longitude=0  Date=2023-01-01  Time=10:30:00  GeoTimeZone=-5.0  SunDaylightSaving=off  wind=0  clouds=10  EnableVolumetricClouds=off  CloudCoverage=0  CloudAltitude=6  fog=0  rain=0  RaindropsEffect=off  SnowDensity=0  EnableGeospatial=off  TilesetSource=Earth terrain  UseTrueOrigin=off  OriginHeight=200  OriginLatitude=40.744652  OriginLongitude=-73.988864  MapStyle=Aerial  AdditionalAssetIDs=[]  UseAdvancedSunSky=off  SolarTime=11  TimeZone=-5  Day=21  Month=9  Year=2022  UseDaylightSavingTime=on  DSTStartDay=10  DSTStartMonth=3  DSTEndDay=3  DSTEndMonth=11  DSTSwitchHour=2  sensorTag=MainCamera1  sensorId=1  sensorName=MainCamera1  mountLoc=Origin  offsetFlag=off  tmountOffset=[0, 0, 0]  rmountOffset=[0, 0, 0]  HorizontalResolution=1280  VerticalResolution=720  HorizontalFOV=60  mountPoint=[0 0 0]  mountOrientation=[0 0 0]  aMode=0  ID=1  GeoTrigger=Inactive  ViewNameList={'Custom'}  ViewTranslationList={'[-1500 0 500]'}  ViewRotationList={'[0 0 0]'}
      settings: AttributesFormatString=ICRF  LibrarySourceBlock=aerolibsim3d/Simulation 3D Scene Configuration
  Subsystem1 : Subsystem
  Subsystem2 : Subsystem
  Transpose : Math  Commented=on  Operator=transpose
  Transpose3 : Math  Commented=on  Operator=transpose
  q : Scope
  tau : Scope  NumInputPorts=3
      settings: ActiveDisplayYMinimum=-0.047636494414562428  ActiveDisplayYMaximum=0.060516242533250761  DataLoggingVariableName=ScopeData2
  actual_ephem : Outport
  actual_ads : Outport  Port=2
  mode_degraded : Outport  Port=3
  wires:
  ads_fault/1 -> Subsystem1/5(ads_fault)
  gps_valid/1 -> Subsystem1/2(gps_valid)
  mission_cmd/1 -> Subsystem1/1(mission_cmd)
  tle_error_high/1 -> Subsystem1/3(tle_error_high)
  ads_fine_allowed/1 -> Subsystem1/4(ads_fine_allowed)
  reference_available/1 -> Subsystem1/6(reference_available)
  energy_low/1 -> Subsystem1/7(energy_low)
  recovery_ready/1 -> Subsystem1/8(recovery_ready)
  optical_target_available/1 -> Subsystem1/11(optical_target_available)
  spin_axis_available/1 -> Subsystem1/10(spin_axis_available)
  spin_feasible/1 -> Subsystem1/9(spin_feasible)
  sun_sensor_valid/1 -> Subsystem1/12(sun_sensor_valid)
  intersat_sensor_tracking/1 -> Subsystem1/13(intersat_sensor_tracking)
  Actuator models/2(RW_omega) -> Subsystem1/17(RW_omega), Scope/1
  Subsystem1/1(actual_ephem) -> actual_ephem/1
  Subsystem1/2(actual_ads) -> actual_ads/1
  Subsystem1/3(mode_degraded) -> mode_degraded/1
  Subsystem1/4(RW_tau) -> tau/3, Actuator models/5(RW_tau)
  Subsystem1/5(THR_tau) -> tau/2, Actuator models/4(THR_tau)
  Subsystem1/6(MTQ_tau) -> Actuator models/3(MTQ_tau), tau/1
  Constant/1 -> Subsystem1/16(B), Actuator models/2(B)
  Transpose/1 -> Simulation 3D Actor/1
  Quaternions to Rotation Angles/1 -> Transpose/1
  Actuator models/1(tau_total) -> Attitude Dynamics/3
  Attitude Dynamics/1 -> Subsystem1/14(q_BI), Quaternions to Rotation Angles/1, q/1
  Attitude Dynamics/2 -> Subsystem1/15(omega), Actuator models/1(omega), Transpose3/1
  Transpose3/1 -> Simulation 3D Actor/2
  Orbit Position/1 -> Attitude Dynamics/1
  Orbit Velocity/1 -> Attitude Dynamics/2

== system ADCS_v1/Actuator models ==
  omega : Inport
  B : Inport  Port=2
  MTQ_tau : Inport  Port=3
  THR_tau : Inport  Port=4
  RW_tau : Inport  Port=5
  Cross Product : matrix_library/Cross Product
  Gain : Gain  Gain=-1
  Gain1 : Gain  Gain=-1
  Gain2 : Gain  Gain=-1
  RW model : Subsystem
  Sum : Sum  Inputs=+++
  tau_total : Outport
  RW_omega : Outport  Port=2
  wires:
  omega/1 -> RW model/1(w)
  RW_tau/1 -> Gain1/1
  RW model/2(hw) -> RW_omega/1
  B/1 -> Cross Product/2
  MTQ_tau/1 -> Gain2/1
  Sum/1 -> tau_total/1
  Cross Product/1 -> Sum/1
  THR_tau/1 -> Gain/1
  RW model/1(tau) -> Sum/2
  Gain/1 -> Sum/3
  Gain1/1 -> RW model/2(tau_cmd)
  Gain2/1 -> Cross Product/1

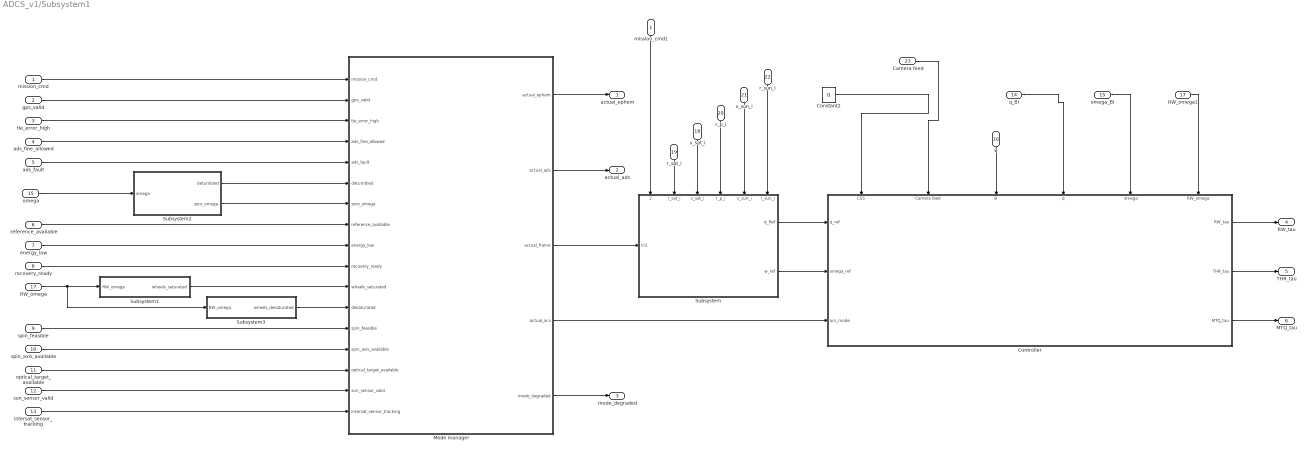
== system ADCS_v1/Subsystem1 ==
  mission_cmd : Inport
  gps_valid : Inport  Port=2
  tle_error_high : Inport  Port=3
  ads_fine_allowed : Inport  Port=4
  ads_fault : Inport  Port=5
  reference_available : Inport  Port=6
  energy_low : Inport  Port=7
  recovery_ready : Inport  Port=8
  spin_feasible : Inport  Port=9
  spin_axis_available : Inport  Port=10
  optical_target_available : Inport  Port=11
  sun_sensor_valid : Inport  Port=12
  intersat_sensor_tracking : Inport  Port=13
  q_BI : Inport  Port=14
  omega : Inport  Port=15
  B : Inport  Port=16
  RW_omega : Inport  Port=17
  v_sat_i : Inport  Port=18
  r_sat_i : Inport  Port=19
  r_p_i : Inport  Port=20
  v_sun_i : Inport  Port=21
  r_sun_i : Inport  Port=22
  Camera feed : Inport  Port=23
  Constant2 : Constant  Value=0
  Controller : Subsystem
      settings: PortSchema="{\"entries\":[{\"content\":{\"sides\":[{\"content\":{\"connectorIds\":[\"In1\",\"In2\",\"In3\"]},\"type\":\"ConnectorPlacement.EquallySpacedRectSide\",\"uuid\":\"3d0ce77c-a0dd-4e63-bb58-aa259872b360\"},{\"content\":{\"connectorIds\":[\"Out1\",\"Out2\",\"Out3\"],\"side\":\"RIGHT\"},\"type\":\"ConnectorPlacement.EquallySpacedRectSide\",\"uuid\":\"c51ce6d0-00d2-499a-9be1-102c03c9909c\"},{\"content\":{\"connectorIds\":[\"In4\",\"In5\",\"In6\",\"In7\",\"In8\",\"In9\"],\"side\":\"TOP\"},\"type\":\"ConnectorPlacement.EquallySpacedRectSide\",\"uuid\":\"ed1e7bc4-2cca-4611-893f-1128994bf2d9\"},{\"content\":{\"side\":\"BOTTOM\"},\"type\":\"ConnectorPlacement.EquallySpacedRectSide\",\"uuid\":\"574e7f6a-1005-4b0c-82f8-22f1ef6841a8\"}]},\"type\":\"ConnectorPlacement.EquallySpacedConnector\",\"uuid\":\"15c446ec-b512-4968-b865-507fd68d8b0b\"}],\"packageUris\":[\"http://schema.mathworks.com/mf0/Connector/R2020b\"],\"version\":\"1.0\"}"
  Mode manager : Subsystem
  RW_omega1 : InportShadow  Port=17
  Subsystem : Subsystem
      settings: PortSchema="{\"entries\":[{\"content\":{\"sides\":[{\"content\":{\"connectorIds\":[\"In1\"]},\"type\":\"ConnectorPlacement.EquallySpacedRectSide\",\"uuid\":\"74bf1b15-53db-441c-9152-7c9ad8598452\"},{\"content\":{\"connectorIds\":[\"Out1\",\"Out2\"],\"side\":\"RIGHT\"},\"type\":\"ConnectorPlacement.EquallySpacedRectSide\",\"uuid\":\"e98e0885-3f20-4aa1-b3a1-f2c890def05c\"},{\"content\":{\"connectorIds\":[\"In2\",\"In3\",\"In4\",\"In5\",\"In6\",\"In7\"],\"side\":\"TOP\"},\"type\":\"ConnectorPlacement.EquallySpacedRectSide\",\"uuid\":\"f0898a47-7ae2-48e7-af8a-6d6327a5175a\"}]},\"type\":\"ConnectorPlacement.EquallySpacedConnector\",\"uuid\":\"b563a257-d36a-4c1e-a9df-51a9ac9caccd\"}],\"packageUris\":[\"http://schema.mathworks.com/mf0/Connector/R2020b\"],\"version\":\"1.0\"}"
  Subsystem1 : Subsystem
  Subsystem2 : Subsystem
  Subsystem3 : Subsystem
  mission_cmd1 : InportShadow
  omega_BI : InportShadow  Port=15
  actual_ephem : Outport
  actual_ads : Outport  Port=2
  mode_degraded : Outport  Port=3
  RW_tau : Outport  Port=4
  THR_tau : Outport  Port=5
  MTQ_tau : Outport  Port=6
  wires:
  spin_axis_available/1 -> Mode manager/14(spin_axis_available)
  Controller/1(RW_tau) -> RW_tau/1
  Mode manager/1(actual_ephem) -> actual_ephem/1
  Mode manager/5(mode_degraded) -> mode_degraded/1
  Constant2/1 -> Controller/4(CSS)
  gps_valid/1 -> Mode manager/2(gps_valid)
  RW_omega/1 -> Subsystem3/1(RW_omega), Subsystem1/1(RW_omega)
  Subsystem2/1(detumbled) -> Mode manager/6(detumbled)
  Mode manager/2(actual_ads) -> actual_ads/1
  tle_error_high/1 -> Mode manager/3(tle_error_high)
  Controller/3(MTQ_tau) -> MTQ_tau/1
  Mode manager/4(actual_acs) -> Controller/3(acs_mode)
  Subsystem1/1(wheels_saturated) -> Mode manager/11(wheels_saturated)
  sun_sensor_valid/1 -> Mode manager/16(sun_sensor_valid)
  recovery_ready/1 -> Mode manager/10(recovery_ready)
  Subsystem3/1(wheels_desaturated) -> Mode manager/12(desaturated)
  ads_fine_allowed/1 -> Mode manager/4(ads_fine_allowed)
  spin_feasible/1 -> Mode manager/13(spin_feasible)
  ads_fault/1 -> Mode manager/5(ads_fault)
  energy_low/1 -> Mode manager/9(energy_low)
  intersat_sensor_tracking/1 -> Mode manager/17(intersat_sensor_tracking)
  optical_target_available/1 -> Mode manager/15(optical_target_available)
  mission_cmd/1 -> Mode manager/1(mission_cmd)
  omega/1 -> Subsystem2/1(omega)
  reference_available/1 -> Mode manager/8(reference_available)
  Controller/2(THR_tau) -> THR_tau/1
  RW_omega1/1 -> Controller/9(RW_omega)
  omega_BI/1 -> Controller/8(omega)
  B/1 -> Controller/6(B)
  Mode manager/3(actual_frame) -> Subsystem/1(In2)
  Subsystem/1(q_Ref) -> Controller/1(q_ref)
  Subsystem/2(w_ref) -> Controller/2(omega_ref)
  v_sat_i/1 -> Subsystem/4(v_sat_i)
  r_sat_i/1 -> Subsystem/3(r_sat_i)
  r_p_i/1 -> Subsystem/5(r_p_i)
  v_sun_i/1 -> Subsystem/6(v_sun_i)
  r_sun_i/1 -> Subsystem/7(r_sun_i)
  Subsystem2/2(zero_omega) -> Mode manager/7(zero_omega)
  q_BI/1 -> Controller/7(q)
  Camera feed/1 -> Controller/5(Camera feed)
  mission_cmd1/1 -> Subsystem/2(mission_cmd)

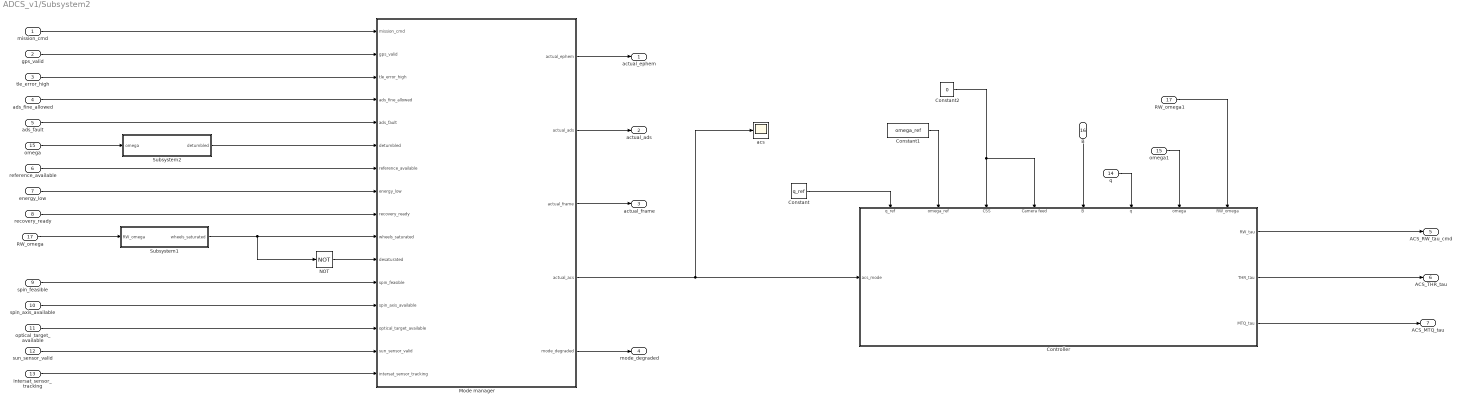
== system ADCS_v1/Subsystem2 ==
  mission_cmd : Inport
  gps_valid : Inport  Port=2
  tle_error_high : Inport  Port=3
  ads_fine_allowed : Inport  Port=4
  ads_fault : Inport  Port=5
  reference_available : Inport  Port=6
  energy_low : Inport  Port=7
  recovery_ready : Inport  Port=8
  spin_feasible : Inport  Port=9
  spin_axis_available : Inport  Port=10
  optical_target_available : Inport  Port=11
  sun_sensor_valid : Inport  Port=12
  intersat_sensor_tracking : Inport  Port=13
  q : Inport  Port=14
  omega : Inport  Port=15
  B : Inport  Port=16
  RW_omega : Inport  Port=17
  Constant : Constant  Value=q_ref
  Constant1 : Constant  Value=omega_ref
  Constant2 : Constant  Value=0
  Controller : Subsystem
      settings: PortSchema="{\"entries\":[{\"content\":{\"sides\":[{\"content\":{\"connectorIds\":[\"In1\"]},\"type\":\"ConnectorPlacement.EquallySpacedRectSide\",\"uuid\":\"3d0ce77c-a0dd-4e63-bb58-aa259872b360\"},{\"content\":{\"connectorIds\":[\"Out1\",\"Out2\",\"Out3\"],\"side\":\"RIGHT\"},\"type\":\"ConnectorPlacement.EquallySpacedRectSide\",\"uuid\":\"c51ce6d0-00d2-499a-9be1-102c03c9909c\"},{\"content\":{\"connectorIds\":[\"In2\",\"In3\",\"In4\",\"In5\",\"In6\",\"In7\",\"In8\",\"In9\"],\"side\":\"TOP\"},\"type\":\"ConnectorPlacement.EquallySpacedRectSide\",\"uuid\":\"ed1e7bc4-2cca-4611-893f-1128994bf2d9\"},{\"content\":{\"side\":\"BOTTOM\"},\"type\":\"ConnectorPlacement.EquallySpacedRectSide\",\"uuid\":\"574e7f6a-1005-4b0c-82f8-22f1ef6841a8\"}]},\"type\":\"ConnectorPlacement.EquallySpacedConnector\",\"uuid\":\"15c446ec-b512-4968-b865-507fd68d8b0b\"}],\"packageUris\":[\"http://schema.mathworks.com/mf0/Connector/R2020b\"],\"version\":\"1.0\"}"
  Mode manager : Subsystem
  NOT : Logic  Operator=NOT  IconShape=distinctive  AllPortsSameDT=off  OutDataTypeStr=boolean
  RW_omega1 : InportShadow  Port=17
  Subsystem1 : Subsystem
  Subsystem2 : Subsystem
  acs : Scope
      settings: ActiveDisplayYMinimum=-1  ActiveDisplayYMaximum=1  DataLoggingVariableName=ScopeData3
  omega1 : InportShadow  Port=15
  actual_ephem : Outport
  actual_ads : Outport  Port=2
  actual_frame : Outport  Port=3
  mode_degraded : Outport  Port=4
  ACS_RW_tau_cmd : Outport  Port=5
  ACS_THR_tau : Outport  Port=6
  ACS_MTQ_tau : Outport  Port=7
  wires:
  B/1 -> Controller/6(B)
  omega1/1 -> Controller/8(omega)
  RW_omega1/1 -> Controller/9(RW_omega)
  Controller/2(THR_tau) -> ACS_THR_tau/1
  reference_available/1 -> Mode manager/7(reference_available)
  omega/1 -> Subsystem2/1(omega)
  mission_cmd/1 -> Mode manager/1(mission_cmd)
  optical_target_available/1 -> Mode manager/14(optical_target_available)
  intersat_sensor_tracking/1 -> Mode manager/16(intersat_sensor_tracking)
  energy_low/1 -> Mode manager/8(energy_low)
  ads_fault/1 -> Mode manager/5(ads_fault)
  spin_feasible/1 -> Mode manager/12(spin_feasible)
  ads_fine_allowed/1 -> Mode manager/4(ads_fine_allowed)
  NOT/1 -> Mode manager/11(desaturated)
  recovery_ready/1 -> Mode manager/9(recovery_ready)
  sun_sensor_valid/1 -> Mode manager/15(sun_sensor_valid)
  Mode manager/3(actual_frame) -> actual_frame/1
  Subsystem1/1(wheels_saturated) -> Mode manager/10(wheels_saturated), NOT/1
  Mode manager/4(actual_acs) -> acs/1, Controller/1(acs_mode)
  Controller/3(MTQ_tau) -> ACS_MTQ_tau/1
  tle_error_high/1 -> Mode manager/3(tle_error_high)
  Mode manager/2(actual_ads) -> actual_ads/1
  Subsystem2/1(detumbled) -> Mode manager/6(detumbled)
  q/1 -> Controller/7(q)
  Constant1/1 -> Controller/3(omega_ref)
  RW_omega/1 -> Subsystem1/1(RW_omega)
  gps_valid/1 -> Mode manager/2(gps_valid)
  Constant2/1 -> Controller/4(CSS), Controller/5(Camera feed)
  Mode manager/5(mode_degraded) -> mode_degraded/1
  Mode manager/1(actual_ephem) -> actual_ephem/1
  Controller/1(RW_tau) -> ACS_RW_tau_cmd/1
  spin_axis_available/1 -> Mode manager/13(spin_axis_available)
  Constant/1 -> Controller/2(q_ref)

== system ADCS_v1/Actuator models/RW model ==
  w : Inport
  tau_cmd : Inport  Port=2
  Abs : Abs  SaturateOnIntegerOverflow=off
  Constant : Constant
  Cross Product : matrix_library/Cross Product
  Gain : Gain  Gain=-1
  Product : Product
  RW torque limit : Saturate  UpperLimit=P.rw.torque_max  LowerLimit=-P.rw.torque_max
  Sum : Sum  Inputs=|++
  Sum1 : Sum  Inputs=|++
  wheel momentum : Integrator  InitialCondition=[0 0 0]  LimitOutput=on  UpperSaturationLimit=P.rw.h_max  LowerSaturationLimit=-P.rw.h_max  ShowSaturationPort=on
  wheel momentum rate : Gain  Gain=-1
  tau : Outport
  hw : Outport  Port=2
  wires:
  Abs/1 -> Gain/1
  wheel momentum rate/1 -> wheel momentum/1
  RW torque limit/1 -> Product/2, wheel momentum rate/1
  wheel momentum/1 -> Cross Product/1, hw/1
  wheel momentum/2 -> Abs/1
  Gain/1 -> Sum/1
  Constant/1 -> Sum/2
  Sum/1 -> Product/1
  tau_cmd/1 -> RW torque limit/1
  Product/1 -> Sum1/2
  w/1 -> Cross Product/2
  Cross Product/1 -> Sum1/1
  Sum1/1 -> tau/1

== system ADCS_v1/Subsystem1/Controller ==
  q_ref : Inport
  omega_ref : Inport  Port=2
  acs_mode : Inport  Port=3
  CSS : Inport  Port=4
  Camera feed : Inport  Port=5
  B : Inport  Port=6
  q : Inport  Port=7
  omega : Inport  Port=8
  RW_omega : Inport  Port=9
  Control Algorithms : Subsystem
  "error " : Subsystem
  omega1 : InportShadow  Port=8
  RW_tau : Outport
  THR_tau : Outport  Port=2
  MTQ_tau : Outport  Port=3
  wires:
  "error "/1(q_err) -> Control Algorithms/7(q_err)
  RW_omega/1 -> Control Algorithms/4(RW_omega)
  CSS/1 -> Control Algorithms/2(CSS)
  Camera feed/1 -> Control Algorithms/5(Camera feed)
  omega/1 -> Control Algorithms/3(omega)
  B/1 -> Control Algorithms/6(B)
  "error "/2(omega_err) -> Control Algorithms/8(omega_err)
  Control Algorithms/1(THR_tau) -> THR_tau/1
  Control Algorithms/2(MTQ_tau) -> MTQ_tau/1
  Control Algorithms/3(RW_tau) -> RW_tau/1
  q_ref/1 -> "error "/1(q_ref)
  q/1 -> "error "/2(q_BI)
  omega_ref/1 -> "error "/3(omega_ref)
  omega1/1 -> "error "/4(omega)
  acs_mode/1 -> Control Algorithms/1(acs_mode)

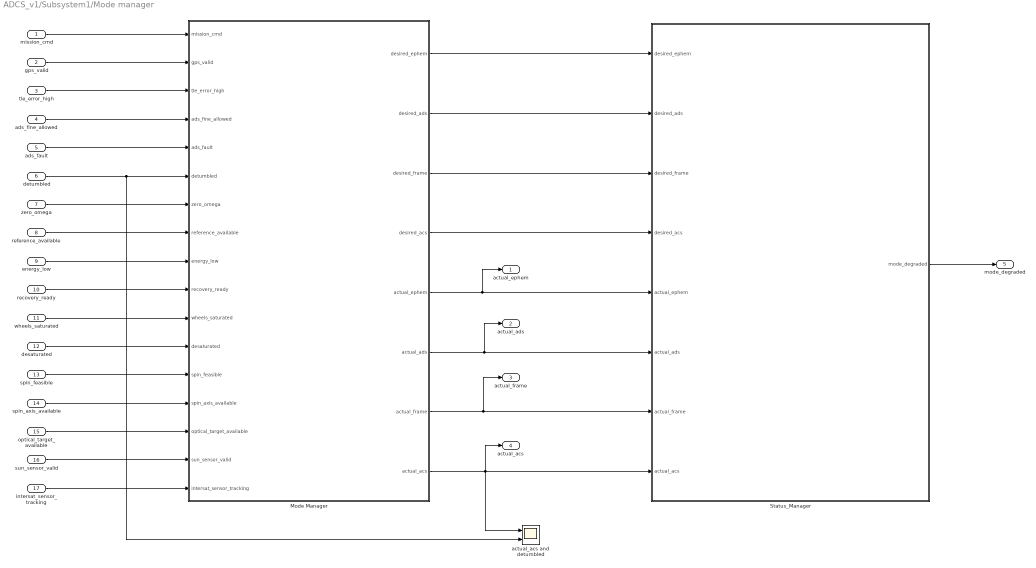
== system ADCS_v1/Subsystem1/Mode manager ==
  mission_cmd : Inport
  gps_valid : Inport  Port=2
  tle_error_high : Inport  Port=3
  ads_fine_allowed : Inport  Port=4
  ads_fault : Inport  Port=5
  detumbled : Inport  Port=6
  zero_omega : Inport  Port=7
  reference_available : Inport  Port=8
  energy_low : Inport  Port=9
  recovery_ready : Inport  Port=10
  wheels_saturated : Inport  Port=11
  desaturated : Inport  Port=12
  spin_feasible : Inport  Port=13
  spin_axis_available : Inport  Port=14
  optical_target_available : Inport  Port=15
  sun_sensor_valid : Inport  Port=16
  intersat_sensor_tracking : Inport  Port=17
  Mode Manager : Subsystem
  Status_Manager : Stateflow chart  TreatAsAtomicUnit=on
  actual_acs and detumbled : Scope  NumInputPorts=2
      settings: ActiveDisplayYMinimum=-0.74999999999999978  ActiveDisplayYMaximum=6.75  DataLoggingVariableName=ScopeData3
  actual_ephem : Outport
  actual_ads : Outport  Port=2
  actual_frame : Outport  Port=3
  actual_acs : Outport  Port=4
  mode_degraded : Outport  Port=5
  wires:
  recovery_ready/1 -> Mode Manager/10(recovery_ready)
  Mode Manager/2(desired_ads) -> Status_Manager/2(desired_ads)
  Mode Manager/8(actual_acs) -> actual_acs/1, Status_Manager/8(actual_acs), actual_acs and detumbled/1
  Mode Manager/1(desired_ephem) -> Status_Manager/1(desired_ephem)
  Mode Manager/5(actual_ephem) -> actual_ephem/1, Status_Manager/5(actual_ephem)
  Mode Manager/6(actual_ads) -> actual_ads/1, Status_Manager/6(actual_ads)
  Mode Manager/7(actual_frame) -> actual_frame/1, Status_Manager/7(actual_frame)
  Mode Manager/3(desired_frame) -> Status_Manager/3(desired_frame)
  Mode Manager/4(desired_acs) -> Status_Manager/4(desired_acs)
  reference_available/1 -> Mode Manager/8(reference_available)
  mission_cmd/1 -> Mode Manager/1(mission_cmd)
  ads_fault/1 -> Mode Manager/5(ads_fault)
  ads_fine_allowed/1 -> Mode Manager/4(ads_fine_allowed)
  wheels_saturated/1 -> Mode Manager/11(wheels_saturated)
  optical_target_available/1 -> Mode Manager/15(optical_target_available)
  detumbled/1 -> Mode Manager/6(detumbled), actual_acs and detumbled/2
  intersat_sensor_tracking/1 -> Mode Manager/17(intersat_sensor_tracking)
  desaturated/1 -> Mode Manager/12(desaturated)
  spin_feasible/1 -> Mode Manager/13(spin_feasible)
  tle_error_high/1 -> Mode Manager/3(tle_error_high)
  energy_low/1 -> Mode Manager/9(energy_low)
  Status_Manager/1(mode_degraded) -> mode_degraded/1
  spin_axis_available/1 -> Mode Manager/14(spin_axis_available)
  sun_sensor_valid/1 -> Mode Manager/16(sun_sensor_valid)
  gps_valid/1 -> Mode Manager/2(gps_valid)
  zero_omega/1 -> Mode Manager/7(zero_omega)

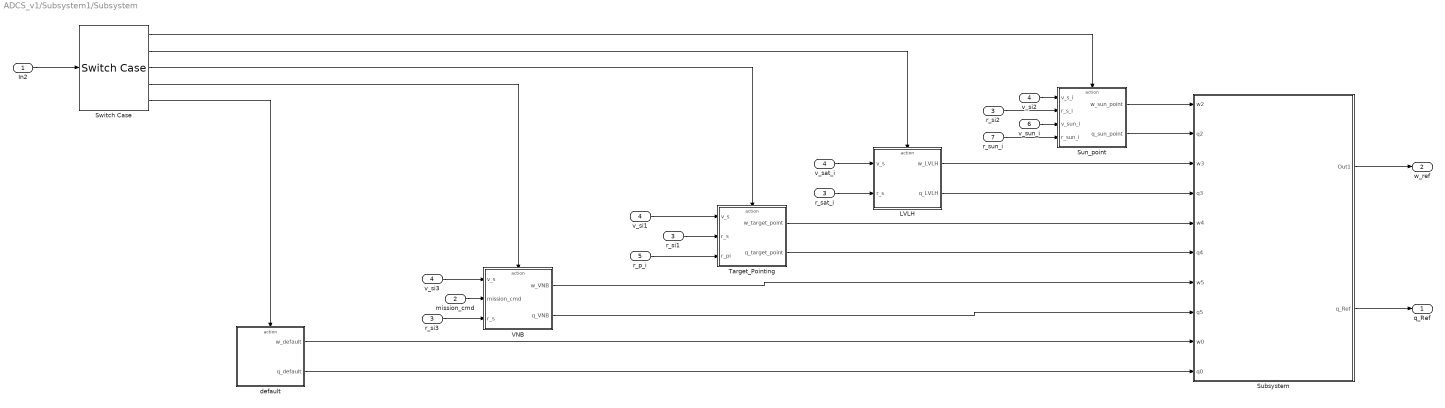
== system ADCS_v1/Subsystem1/Subsystem ==
  In2 : Inport
  mission_cmd : Inport  Port=2
  r_sat_i : Inport  Port=3
  v_sat_i : Inport  Port=4
  r_p_i : Inport  Port=5
  v_sun_i : Inport  Port=6
  r_sun_i : Inport  Port=7
  LVLH : Subsystem
  Subsystem : Subsystem
  Sun_point : Subsystem
  Switch Case : SwitchCase  CaseConditions={2,3,4,5}
  Target_Pointing : Subsystem
  VNB : Subsystem
  default : Subsystem
  r_si1 : InportShadow  Port=3
  r_si2 : InportShadow  Port=3
  r_si3 : InportShadow  Port=3
  v_si1 : InportShadow  Port=4
  v_si2 : InportShadow  Port=4
  v_si3 : InportShadow  Port=4
  q_Ref : Outport
  w_ref : Outport  Port=2
  wires:
  Switch Case/5 -> default/Action
  In2/1 -> Switch Case/1
  r_si1/1 -> Target_Pointing/2(r_s)
  v_si1/1 -> Target_Pointing/1(v_s)
  LVLH/1(w_LVLH) -> Subsystem/3(w3)
  LVLH/2(q_LVLH) -> Subsystem/4(q3)
  Target_Pointing/1(w_target_point) -> Subsystem/5(w4)
  Target_Pointing/2(q_target_point) -> Subsystem/6(q4)
  default/1(w_default) -> Subsystem/9(w0)
  default/2(q_default) -> Subsystem/10(q0)
  Subsystem/1(Out1) -> w_ref/1
  v_sat_i/1 -> LVLH/1(v_s)
  r_sat_i/1 -> LVLH/2(r_s)
  v_si2/1 -> Sun_point/1(v_s_i)
  r_si2/1 -> Sun_point/2(r_s_i)
  Sun_point/1(w_sun_point) -> Subsystem/1(w2)
  Sun_point/2(q_sun_point) -> Subsystem/2(q2)
  r_p_i/1 -> Target_Pointing/3(r_pi)
  v_sun_i/1 -> Sun_point/3(v_sun_i)
  r_sun_i/1 -> Sun_point/4(r_sun_i)
  Switch Case/1 -> Sun_point/Action
  Switch Case/2 -> LVLH/Action
  Switch Case/3 -> Target_Pointing/Action
  Subsystem/2(q_Ref) -> q_Ref/1
  r_si3/1 -> VNB/3(r_s)
  v_si3/1 -> VNB/1(v_s)
  VNB/2(q_VNB) -> Subsystem/8(q5)
  VNB/1(w_VNB) -> Subsystem/7(w5)
  Switch Case/4 -> VNB/Action
  mission_cmd/1 -> VNB/2(mission_cmd)

== system ADCS_v1/Subsystem1/Subsystem1 ==
  RW_omega : Inport
  Abs : Abs  SaturateOnIntegerOverflow=off
  Compare To Constant : simulink/Logic and Bit Operations/Compare To Constant  relop=>=  const=h_max*0.95  OutDataTypeStr=boolean
  Gain : Gain  Gain=I_RW
  Max of Elements : MinMax  Function=max
  wheels_saturated : Outport
  wires:
  Gain/1 -> Compare To Constant/1
  Abs/1 -> Max of Elements/1
  RW_omega/1 -> Abs/1
  Max of Elements/1 -> Gain/1
  Compare To Constant/1 -> wheels_saturated/1

== system ADCS_v1/Subsystem1/Subsystem2 ==
  omega : Inport
  Compare To Constant : simulink/Logic and Bit Operations/Compare To Constant  relop=<=  const=omega_thr^2  OutDataTypeStr=boolean
  Compare To Constant1 : simulink/Logic and Bit Operations/Compare To Constant  relop=<=  const=omega_zero^2  OutDataTypeStr=boolean
  Dot Product : DotProduct  OutDataTypeStr=Inherit: Inherit via internal rule
  detumbled : Outport
  zero_omega : Outport  Port=2
  wires:
  Compare To Constant/1 -> detumbled/1
  omega/1 -> Dot Product/2, Dot Product/1
  Dot Product/1 -> Compare To Constant1/1, Compare To Constant/1
  Compare To Constant1/1 -> zero_omega/1

== system ADCS_v1/Subsystem1/Subsystem3 ==
  RW_omega : Inport
  Abs : Abs  SaturateOnIntegerOverflow=off
  Compare To Constant : simulink/Logic and Bit Operations/Compare To Constant  relop=<=  const=h_max*0.25  OutDataTypeStr=boolean
  Gain : Gain  Gain=I_RW
  Max of Elements : MinMax  Function=max
  wheels_desaturated : Outport
  wires:
  Compare To Constant/1 -> wheels_desaturated/1
  Max of Elements/1 -> Gain/1
  RW_omega/1 -> Abs/1
  Abs/1 -> Max of Elements/1
  Gain/1 -> Compare To Constant/1

== system ADCS_v1/Subsystem2/Controller ==
  acs_mode : Inport
  q_ref : Inport  Port=2
  omega_ref : Inport  Port=3
  CSS : Inport  Port=4
  Camera feed : Inport  Port=5
  B : Inport  Port=6
  q : Inport  Port=7
  omega : Inport  Port=8
  RW_omega : Inport  Port=9
  Control Algorithms : Subsystem
  Subsystem : Subsystem
  omega1 : InportShadow  Port=8
  RW_tau : Outport
  THR_tau : Outport  Port=2
  MTQ_tau : Outport  Port=3
  wires:
  acs_mode/1 -> Control Algorithms/1(acs_mode)
  omega1/1 -> Subsystem/4(omega)
  omega_ref/1 -> Subsystem/3(omega_ref)
  q/1 -> Subsystem/2(q)
  q_ref/1 -> Subsystem/1(q_ref)
  Control Algorithms/3(RW_tau) -> RW_tau/1
  Control Algorithms/2(MTQ_tau) -> MTQ_tau/1
  Control Algorithms/1(THR_tau) -> THR_tau/1
  Subsystem/2(omega_err) -> Control Algorithms/8(omega_err)
  B/1 -> Control Algorithms/6(B)
  omega/1 -> Control Algorithms/3(omega)
  Camera feed/1 -> Control Algorithms/5(Camera feed)
  CSS/1 -> Control Algorithms/2(CSS)
  RW_omega/1 -> Control Algorithms/4(RW_omega)
  Subsystem/1(q_err) -> Control Algorithms/7(q_err)

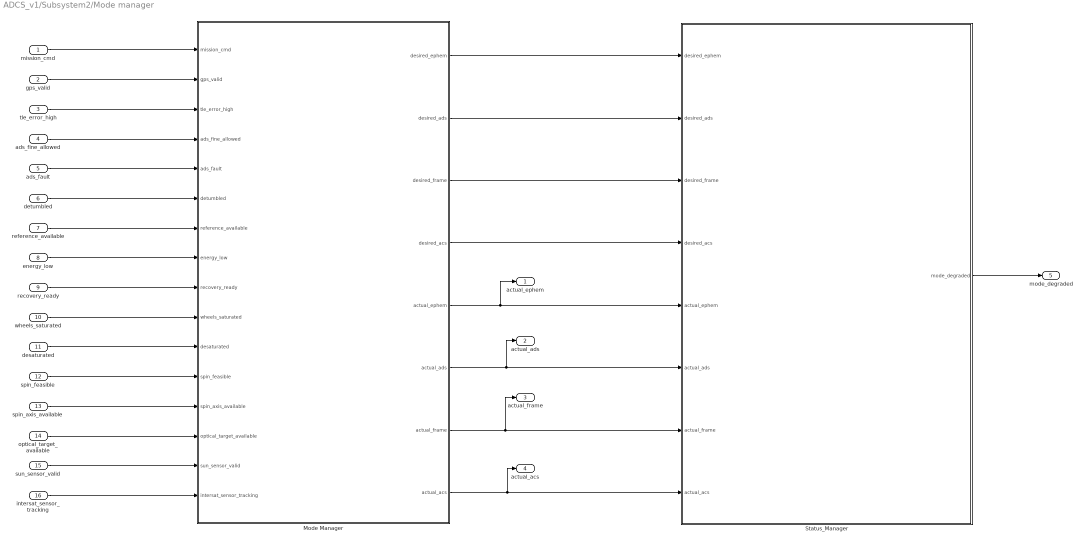
== system ADCS_v1/Subsystem2/Mode manager ==
  mission_cmd : Inport
  gps_valid : Inport  Port=2
  tle_error_high : Inport  Port=3
  ads_fine_allowed : Inport  Port=4
  ads_fault : Inport  Port=5
  detumbled : Inport  Port=6
  reference_available : Inport  Port=7
  energy_low : Inport  Port=8
  recovery_ready : Inport  Port=9
  wheels_saturated : Inport  Port=10
  desaturated : Inport  Port=11
  spin_feasible : Inport  Port=12
  spin_axis_available : Inport  Port=13
  optical_target_available : Inport  Port=14
  sun_sensor_valid : Inport  Port=15
  intersat_sensor_tracking : Inport  Port=16
  Mode Manager : Subsystem
  Status_Manager : Stateflow chart  TreatAsAtomicUnit=on
  actual_ephem : Outport
  actual_ads : Outport  Port=2
  actual_frame : Outport  Port=3
  actual_acs : Outport  Port=4
  mode_degraded : Outport  Port=5
  wires:
  gps_valid/1 -> Mode Manager/2(gps_valid)
  sun_sensor_valid/1 -> Mode Manager/15(sun_sensor_valid)
  spin_axis_available/1 -> Mode Manager/13(spin_axis_available)
  Status_Manager/1(mode_degraded) -> mode_degraded/1
  energy_low/1 -> Mode Manager/8(energy_low)
  tle_error_high/1 -> Mode Manager/3(tle_error_high)
  spin_feasible/1 -> Mode Manager/12(spin_feasible)
  desaturated/1 -> Mode Manager/11(desaturated)
  intersat_sensor_tracking/1 -> Mode Manager/16(intersat_sensor_tracking)
  detumbled/1 -> Mode Manager/6(detumbled)
  optical_target_available/1 -> Mode Manager/14(optical_target_available)
  wheels_saturated/1 -> Mode Manager/10(wheels_saturated)
  ads_fine_allowed/1 -> Mode Manager/4(ads_fine_allowed)
  ads_fault/1 -> Mode Manager/5(ads_fault)
  mission_cmd/1 -> Mode Manager/1(mission_cmd)
  reference_available/1 -> Mode Manager/7(reference_available)
  Mode Manager/4(desired_acs) -> Status_Manager/4(desired_acs)
  Mode Manager/3(desired_frame) -> Status_Manager/3(desired_frame)
  Mode Manager/7(actual_frame) -> Status_Manager/7(actual_frame), actual_frame/1
  Mode Manager/6(actual_ads) -> Status_Manager/6(actual_ads), actual_ads/1
  Mode Manager/5(actual_ephem) -> Status_Manager/5(actual_ephem), actual_ephem/1
  Mode Manager/1(desired_ephem) -> Status_Manager/1(desired_ephem)
  Mode Manager/8(actual_acs) -> Status_Manager/8(actual_acs), actual_acs/1
  Mode Manager/2(desired_ads) -> Status_Manager/2(desired_ads)
  recovery_ready/1 -> Mode Manager/9(recovery_ready)

== system ADCS_v1/Subsystem2/Subsystem1 ==
  RW_omega : Inport
  Abs : Abs  SaturateOnIntegerOverflow=off
  Compare To Constant : simulink/Logic and Bit Operations/Compare To Constant  relop=<=  const=h_max  OutDataTypeStr=boolean
  Gain : Gain  Gain=I_RW
  Max of Elements : MinMax  Function=max
  wheels_saturated : Outport
  wires:
  Compare To Constant/1 -> wheels_saturated/1
  Max of Elements/1 -> Gain/1
  RW_omega/1 -> Abs/1
  Abs/1 -> Max of Elements/1
  Gain/1 -> Compare To Constant/1

== system ADCS_v1/Subsystem2/Subsystem2 ==
  omega : Inport
  Compare To Constant : simulink/Logic and Bit Operations/Compare To Constant  relop=<=  const=omega_thr^2  OutDataTypeStr=boolean
  Dot Product : DotProduct  OutDataTypeStr=Inherit: Inherit via internal rule
  detumbled : Outport
  wires:
  Dot Product/1 -> Compare To Constant/1
  omega/1 -> Dot Product/1, Dot Product/2
  Compare To Constant/1 -> detumbled/1

== system ADCS_v1/Subsystem1/Controller/Control Algorithms ==
  acs_mode : Inport
  CSS : Inport  Port=2
  omega : Inport  Port=3
  RW_omega : Inport  Port=4
  Camera feed : Inport  Port=5
  B : Inport  Port=6
  q_err : Inport  Port=7
  omega_err : Inport  Port=8
  DESAT : Subsystem  TreatAsAtomicUnit=on
  Gain : Gain  Gain=0
  Merge : Merge
  RW Torque Commands : Subsystem
      settings: PortSchema="{\"entries\":[{\"content\":{\"sides\":[{\"content\":{\"connectorIds\":[\"In1\",\"In2\",\"In3\",\"In4\",\"In5\",\"In6\",\"In7\",\"In8\"]},\"type\":\"ConnectorPlacement.EquallySpacedRectSide\",\"uuid\":\"3d0ce77c-a0dd-4e63-bb58-aa259872b360\"},{\"content\":{\"connectorIds\":[\"Out1\"],\"side\":\"RIGHT\"},\"type\":\"ConnectorPlacement.EquallySpacedRectSide\",\"uuid\":\"c51ce6d0-00d2-499a-9be1-102c03c9909c\"},{\"content\":{\"connectorIds\":[\"In9\",\"In10\"],\"side\":\"TOP\"},\"type\":\"ConnectorPlacement.EquallySpacedRectSide\",\"uuid\":\"ed1e7bc4-2cca-4611-893f-1128994bf2d9\"}]},\"type\":\"ConnectorPlacement.EquallySpacedConnector\",\"uuid\":\"15c446ec-b512-4968-b865-507fd68d8b0b\"}],\"packageUris\":[\"http://schema.mathworks.com/mf0/Connector/R2020b\"],\"version\":\"1.0\"}"
  Switch Case1 : SwitchCase  CaseConditions={1,4}
  Switch Case2 : SwitchCase  CaseConditions={4}
  Switch Case3 : SwitchCase  CaseConditions={2,3,4,5,6}
  Thruster Torque commands : Subsystem
  default : Subsystem  TreatAsAtomicUnit=on
  THR_tau : Outport
  MTQ_tau : Outport  Port=2
  RW_tau : Outport  Port=3
  wires:
  Camera feed/1 -> RW Torque Commands/1(Camera feed)
  RW_omega/1 -> Thruster Torque commands/5(RW_omega), DESAT/2(RW_omega)
  B/1 -> DESAT/1(B)
  CSS/1 -> RW Torque Commands/8(CSS)
  omega/1 -> Thruster Torque commands/4(omega)
  omega_err/1 -> RW Torque Commands/9(omega_err)
  q_err/1 -> RW Torque Commands/10(q_err)
  Switch Case1/1 -> Thruster Torque commands/1(detumble)
  Switch Case1/3 -> Thruster Torque commands/3(default)
  default/1(tau_cmd) -> Merge/2
  Switch Case2/2 -> default/Action
  DESAT/1(tau_cmd) -> Merge/1
  Merge/1 -> Gain/1
  Switch Case2/1 -> DESAT/Action
  Switch Case3/1 -> RW Torque Commands/2(point)
  Switch Case3/2 -> RW Torque Commands/3(spin)
  Switch Case3/3 -> RW Torque Commands/4(desat)
  Switch Case3/6 -> RW Torque Commands/7(idle)
  acs_mode/1 -> Switch Case3/1, Switch Case1/1, Switch Case2/1
  Gain/1 -> MTQ_tau/1
  RW Torque Commands/1(tau_cmd) -> RW_tau/1
  Thruster Torque commands/1(tau_cmd) -> THR_tau/1
  Switch Case1/2 -> Thruster Torque commands/2(desat)
  Switch Case3/4 -> RW Torque Commands/5(optical)
  Switch Case3/5 -> RW Torque Commands/6(safe)

== system ADCS_v1/Subsystem1/Controller/error  ==
  q_ref : Inport
  q_BI : Inport  Port=2
  omega_ref : Inport  Port=3
  omega : Inport  Port=4
  Product : Product  Multiplication=Matrix(*)
  Quaternion Conjugate1 : aerolibutil/Quaternion Conjugate
  Quaternion Multiplication : aerolibutil/Quaternion Multiplication
  Quaternions to Direction Cosine Matrix : Quat2Dcm
  Shortest q error : Switch  SaturateOnIntegerOverflow=off  InputSameDT=off
  Sum : Sum  Inputs=|+-
  Transpose : Math  Operator=transpose
  Transpose1 : Math  Operator=transpose
  q_err sign flip : Gain  Gain=-1
  split q_error : Demux  Outputs=[1 3]
  q_err : Outport
  omega_err : Outport  Port=2
  wires:
  Sum/1 -> omega_err/1
  Quaternion Multiplication/1 -> Quaternion Conjugate1/1
  q_BI/1 -> Quaternions to Direction Cosine Matrix/1, Quaternion Multiplication/2
  omega/1 -> Sum/1
  Shortest q error/1 -> q_err/1
  split q_error/2 -> Shortest q error/1, q_err sign flip/1
  split q_error/1 -> Shortest q error/2
  q_err sign flip/1 -> Shortest q error/3
  Quaternions to Direction Cosine Matrix/1 -> Product/1
  Product/1 -> Transpose1/1
  omega_ref/1 -> Transpose/1
  Transpose/1 -> Product/2
  Transpose1/1 -> Sum/2
  Quaternion Conjugate1/1 -> split q_error/1
  q_ref/1 -> Quaternion Multiplication/1

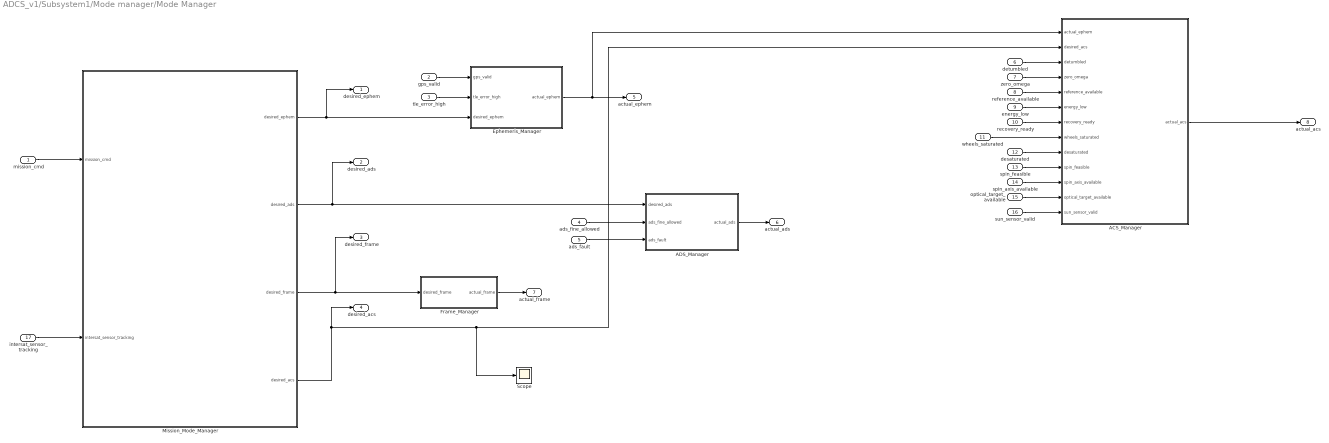
== system ADCS_v1/Subsystem1/Mode manager/Mode Manager ==
  mission_cmd : Inport  OutDataTypeStr=uint8  PortDimensions=1
  gps_valid : Inport  Port=2  OutDataTypeStr=boolean  PortDimensions=1
  tle_error_high : Inport  Port=3  OutDataTypeStr=boolean  PortDimensions=1
  ads_fine_allowed : Inport  Port=4  OutDataTypeStr=boolean  PortDimensions=1
  ads_fault : Inport  Port=5  OutDataTypeStr=boolean  PortDimensions=1
  detumbled : Inport  Port=6  OutDataTypeStr=boolean  PortDimensions=1
  zero_omega : Inport  Port=7
  reference_available : Inport  Port=8  OutDataTypeStr=boolean  PortDimensions=1
  energy_low : Inport  Port=9  OutDataTypeStr=boolean  PortDimensions=1
  recovery_ready : Inport  Port=10  OutDataTypeStr=boolean  PortDimensions=1
  wheels_saturated : Inport  Port=11  OutDataTypeStr=boolean  PortDimensions=1
  desaturated : Inport  Port=12  OutDataTypeStr=boolean  PortDimensions=1
  spin_feasible : Inport  Port=13  OutDataTypeStr=boolean  PortDimensions=1
  spin_axis_available : Inport  Port=14  OutDataTypeStr=boolean  PortDimensions=1
  optical_target_available : Inport  Port=15  OutDataTypeStr=boolean  PortDimensions=1
  sun_sensor_valid : Inport  Port=16  OutDataTypeStr=boolean  PortDimensions=1
  intersat_sensor_tracking : Inport  Port=17  OutDataTypeStr=boolean  PortDimensions=1
  ACS_Manager : Stateflow chart  TreatAsAtomicUnit=on
      settings: PortSchema="{\"entries\":[{\"content\":{\"sides\":[{\"content\":{\"connectorIds\":[\"In2\",\"In1\",\"In3\",\"In4\",\"In5\",\"In6\",\"In7\",\"In8\",\"In9\",\"In10\",\"In11\",\"In12\",\"In13\"]},\"type\":\"ConnectorPlacement.EquallySpacedRectSide\",\"uuid\":\"c64f5ed7-7a07-4761-a251-d625087249f8\"},{\"content\":{\"connectorIds\":[\"Out1\"],\"side\":\"RIGHT\"},\"type\":\"ConnectorPlacement.EquallySpacedRectSide\",\"uuid\":\"ff17dfa7-5a32-4799-bec0-131df3b46d45\"},{\"content\":{\"side\":\"TOP\"},\"type\":\"ConnectorPlacement.EquallySpacedRectSide\",\"uuid\":\"acaf274e-12ec-4fab-ab7e-ad580afcef6e\"},{\"content\":{\"side\":\"BOTTOM\"},\"type\":\"ConnectorPlacement.EquallySpacedRectSide\",\"uuid\":\"23b8eb5a-32b2-43f2-9f21-5c184446e61f\"}]},\"type\":\"ConnectorPlacement.EquallySpacedConnector\",\"uuid\":\"7d19de63-b993-417e-b6e9-9dc888da130b\"}],\"packageUris\":[\"http://schema.mathworks.com/mf0/Connector/R2020b\"],\"version\":\"1.0\"}"
  ADS_Manager : Stateflow chart  TreatAsAtomicUnit=on
  Ephemeris_Manager : Stateflow chart  TreatAsAtomicUnit=on
      settings: PortSchema="{\"entries\":[{\"content\":{\"sides\":[{\"content\":{\"connectorIds\":[\"In2\",\"In3\",\"In1\"]},\"type\":\"ConnectorPlacement.EquallySpacedRectSide\",\"uuid\":\"cbbccf67-8c60-498d-a98a-76db8747fb3a\"},{\"content\":{\"connectorIds\":[\"Out1\"],\"side\":\"RIGHT\"},\"type\":\"ConnectorPlacement.EquallySpacedRectSide\",\"uuid\":\"743b35d2-d398-4833-9c20-93b5e77612f2\"},{\"content\":{\"side\":\"TOP\"},\"type\":\"ConnectorPlacement.EquallySpacedRectSide\",\"uuid\":\"56075cc1-c683-438a-85bf-78d94186ffa6\"}]},\"type\":\"ConnectorPlacement.EquallySpacedConnector\",\"uuid\":\"bae867d4-09fc-4097-a23b-eff5fb3633ac\"}],\"packageUris\":[\"http://schema.mathworks.com/mf0/Connector/R2020b\"],\"version\":\"1.0\"}"
  Frame_Manager : Stateflow chart  TreatAsAtomicUnit=on
  Mission_Mode_Manager : Stateflow chart  TreatAsAtomicUnit=on
  Scope : Scope
      settings: ActiveDisplayYMinimum=-1  ActiveDisplayYMaximum=1  DataLoggingVariableName=ScopeData4
  desired_ephem : Outport
  desired_ads : Outport  Port=2
  desired_frame : Outport  Port=3
  desired_acs : Outport  Port=4
  actual_ephem : Outport  Port=5
  actual_ads : Outport  Port=6
  actual_frame : Outport  Port=7
  actual_acs : Outport  Port=8
  wires:
  sun_sensor_valid/1 -> ACS_Manager/13(sun_sensor_valid)
  ACS_Manager/1(actual_acs) -> actual_acs/1
  Mission_Mode_Manager/4(desired_acs) -> Scope/1, ACS_Manager/1(desired_acs), desired_acs/1
  energy_low/1 -> ACS_Manager/6(energy_low)
  Mission_Mode_Manager/1(desired_ephem) -> Ephemeris_Manager/1(desired_ephem), desired_ephem/1
  Frame_Manager/1(actual_frame) -> actual_frame/1
  optical_target_available/1 -> ACS_Manager/12(optical_target_available)
  Mission_Mode_Manager/2(desired_ads) -> desired_ads/1, ADS_Manager/1(desired_ads)
  tle_error_high/1 -> Ephemeris_Manager/3(tle_error_high)
  reference_available/1 -> ACS_Manager/5(reference_available)
  detumbled/1 -> ACS_Manager/3(detumbled)
  wheels_saturated/1 -> ACS_Manager/8(wheels_saturated)
  Mission_Mode_Manager/3(desired_frame) -> desired_frame/1, Frame_Manager/1(desired_frame)
  ADS_Manager/1(actual_ads) -> actual_ads/1
  ads_fine_allowed/1 -> ADS_Manager/2(ads_fine_allowed)
  Ephemeris_Manager/1(actual_ephem) -> actual_ephem/1, ACS_Manager/2(actual_ephem)
  gps_valid/1 -> Ephemeris_Manager/2(gps_valid)
  intersat_sensor_tracking/1 -> Mission_Mode_Manager/2(intersat_sensor_tracking)
  ads_fault/1 -> ADS_Manager/3(ads_fault)
  recovery_ready/1 -> ACS_Manager/7(recovery_ready)
  mission_cmd/1 -> Mission_Mode_Manager/1(mission_cmd)
  spin_axis_available/1 -> ACS_Manager/11(spin_axis_available)
  desaturated/1 -> ACS_Manager/9(desaturated)
  spin_feasible/1 -> ACS_Manager/10(spin_feasible)
  zero_omega/1 -> ACS_Manager/4(zero_omega)

== system ADCS_v1/Subsystem1/Subsystem/LVLH ==
  v_s : Inport
  r_s : Inport  Port=2
  Action Port : ActionPort
  Cross Product : matrix_library/Cross Product
  Cross Product1 : matrix_library/Cross Product
  Direction Cosine Matrix to Quaternions : Dcm2Quat
  Divide : Product  Inputs=*/
  Divide1 : Product  Inputs=*/
  Divide2 : Product  Inputs=*/
  Gain : Gain  Gain=-1
  Mux : Mux  Inputs=3
  Reshape : Reshape  OutputDimensionality=Customize  OutputDimensions=[3,3]
  Scope : Scope
      settings: ActiveDisplayYMinimum=-1  ActiveDisplayYMaximum=1  DataLoggingVariableName=ScopeData6
  Scope1 : Scope
      settings: ActiveDisplayYMinimum=-0.82867069291103368  ActiveDisplayYMaximum=0.87774872275294546
  Square : Math  Operator=square
  Transpose1 : Math  Operator=transpose
  norm : Subsystem
  norm1 : Subsystem
  w_LVLH : Outport
  q_LVLH : Outport  Port=2
  wires:
  Transpose1/1 -> Scope/1, w_LVLH/1
  Divide/1 -> Gain/1
  Divide1/1 -> Mux/2, Cross Product1/1
  norm1/1(Out1) -> Divide1/2
  Cross Product1/1 -> Mux/1
  Mux/1 -> Reshape/1
  Square/1 -> Divide2/2
  v_s/1 -> Cross Product/1
  r_s/1 -> norm/1(In1), Divide/1, Cross Product/2
  norm/1(Out1) -> Square/1, Divide/2
  Divide2/1 -> Transpose1/1
  Direction Cosine Matrix to Quaternions/1 -> q_LVLH/1, Scope1/1
  Gain/1 -> Mux/3, Cross Product1/2
  Cross Product/1 -> Divide2/1, Divide1/1, norm1/1(In1)
  Reshape/1 -> Direction Cosine Matrix to Quaternions/1

== system ADCS_v1/Subsystem1/Subsystem/Subsystem ==
  w2 : Inport
  q2 : Inport  Port=2
  w3 : Inport  Port=3
  q3 : Inport  Port=4
  w4 : Inport  Port=5
  q4 : Inport  Port=6
  w5 : Inport  Port=7
  q5 : Inport  Port=8
  w0 : Inport  Port=9
  q0 : Inport  Port=10
  Merge : Merge  Inputs=5
  Merge1 : Merge  Inputs=5
  Transpose2 : Math  Operator=transpose
  Out1 : Outport
  q_Ref : Outport  Port=2
  wires:
  q4/1 -> Merge1/3
  q3/1 -> Merge1/2
  Merge/1 -> Transpose2/1
  q2/1 -> Merge1/1
  Merge1/1 -> q_Ref/1
  w4/1 -> Merge/3
  w3/1 -> Merge/2
  w2/1 -> Merge/1
  Transpose2/1 -> Out1/1
  q0/1 -> Merge1/5
  q5/1 -> Merge1/4
  w0/1 -> Merge/5
  w5/1 -> Merge/4

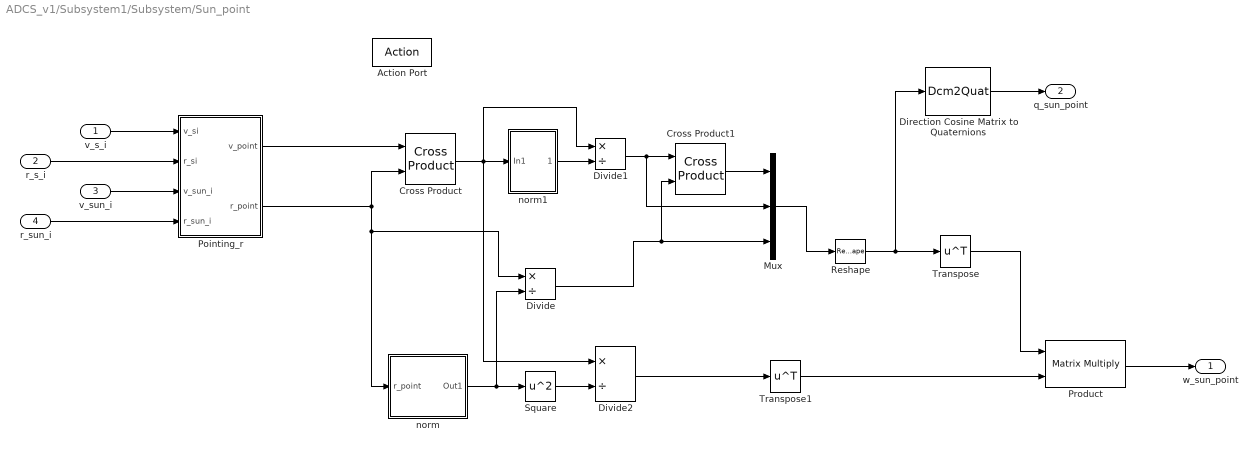
== system ADCS_v1/Subsystem1/Subsystem/Sun_point ==
  v_s_i : Inport
  r_s_i : Inport  Port=2
  v_sun_i : Inport  Port=3
  r_sun_i : Inport  Port=4
  Action Port : ActionPort
  Cross Product : matrix_library/Cross Product
  Cross Product1 : matrix_library/Cross Product
  Direction Cosine Matrix to Quaternions : Dcm2Quat
  Divide : Product  Inputs=*/
  Divide1 : Product  Inputs=*/
  Divide2 : Product  Inputs=*/
  Mux : Mux  Inputs=3
  Pointing_r : Subsystem
  Product : Product  Multiplication=Matrix(*)
  Reshape : Reshape  OutputDimensionality=Customize  OutputDimensions=[3,3]
  Square : Math  Operator=square
  Transpose : Math  Operator=transpose
  Transpose1 : Math  Operator=transpose
  norm : Subsystem
  norm1 : Subsystem
  w_sun_point : Outport
  q_sun_point : Outport  Port=2
  wires:
  Product/1 -> w_sun_point/1
  Direction Cosine Matrix to Quaternions/1 -> q_sun_point/1
  Transpose/1 -> Product/1
  Reshape/1 -> Transpose/1, Direction Cosine Matrix to Quaternions/1
  Transpose1/1 -> Product/2
  Cross Product1/1 -> Mux/1
  Divide/1 -> Cross Product1/2, Mux/3
  Square/1 -> Divide2/2
  norm1/1(Out1) -> Divide1/2
  Divide1/1 -> Mux/2, Cross Product1/1
  Cross Product/1 -> norm1/1(In1), Divide1/1, Divide2/1
  Pointing_r/2(r_point) -> Divide/1, norm/1(r_point), Cross Product/2
  Mux/1 -> Reshape/1
  norm/1(Out1) -> Square/1, Divide/2
  Divide2/1 -> Transpose1/1
  Pointing_r/1(v_point) -> Cross Product/1
  r_s_i/1 -> Pointing_r/2(r_si)
  v_s_i/1 -> Pointing_r/1(v_si)
  v_sun_i/1 -> Pointing_r/3(v_sun_i)
  r_sun_i/1 -> Pointing_r/4(r_sun_i)

== system ADCS_v1/Subsystem1/Subsystem/Target_Pointing ==
  v_s : Inport
  r_s : Inport  Port=2
  r_pi : Inport  Port=3
  Action Port : ActionPort
  Cross Product : matrix_library/Cross Product
  Cross Product1 : matrix_library/Cross Product
  Direction Cosine Matrix to Quaternions : Dcm2Quat
  Divide : Product  Inputs=*/
  Divide1 : Product  Inputs=*/
  Divide2 : Product  Inputs=*/
  Mux : Mux  Inputs=3
  Pointing_r : Subsystem
  Product : Product  Multiplication=Matrix(*)
  Reshape : Reshape  OutputDimensionality=Customize  OutputDimensions=[3,3]
  Square : Math  Operator=square
  Transpose : Math  Operator=transpose
  Transpose1 : Math  Operator=transpose
  norm : Subsystem
  norm1 : Subsystem
  w_target_point : Outport
  q_target_point : Outport  Port=2
  wires:
  v_s/1 -> Pointing_r/1(v_si)
  r_s/1 -> Pointing_r/2(r_si)
  Pointing_r/1(v_point) -> Cross Product/1
  Divide2/1 -> Transpose1/1
  norm/1(Out1) -> Divide/2, Square/1
  Mux/1 -> Reshape/1
  Pointing_r/2(r_point) -> norm/1(r_point), Divide/1, Cross Product/2
  Cross Product/1 -> Divide2/1, Divide1/1, norm1/1(In1)
  Divide1/1 -> Cross Product1/1, Mux/2
  norm1/1(Out1) -> Divide1/2
  Square/1 -> Divide2/2
  Divide/1 -> Mux/3, Cross Product1/2
  Cross Product1/1 -> Mux/1
  Transpose1/1 -> Product/2
  Reshape/1 -> Direction Cosine Matrix to Quaternions/1, Transpose/1
  Transpose/1 -> Product/1
  Direction Cosine Matrix to Quaternions/1 -> q_target_point/1
  Product/1 -> w_target_point/1
  r_pi/1 -> Pointing_r/3(r_pi)

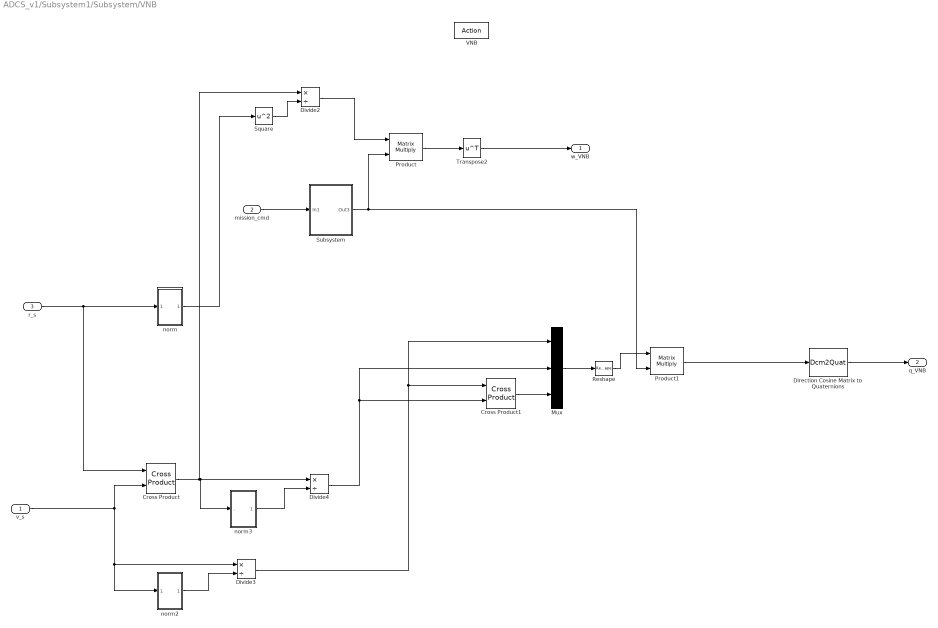
== system ADCS_v1/Subsystem1/Subsystem/VNB ==
  v_s : Inport
  mission_cmd : Inport  Port=2
  r_s : Inport  Port=3
  VNB : ActionPort
  Cross Product : matrix_library/Cross Product
  Cross Product1 : matrix_library/Cross Product
  Direction Cosine Matrix to Quaternions : Dcm2Quat
  Divide2 : Product  Inputs=*/
  Divide3 : Product  Inputs=*/
  Divide4 : Product  Inputs=*/
  Mux : Mux  Inputs=3
  Product : Product  Multiplication=Matrix(*)
  Product1 : Product  Multiplication=Matrix(*)
  Reshape : Reshape  OutputDimensionality=Customize  OutputDimensions=[3,3]
  Square : Math  Operator=square
  Subsystem : Subsystem
  Transpose2 : Math  Operator=transpose
  norm : Subsystem
  norm2 : Subsystem
  norm3 : Subsystem
  w_VNB : Outport
  q_VNB : Outport  Port=2
  wires:
  Product/1 -> Transpose2/1
  Square/1 -> Divide2/2
  r_s/1 -> norm/1(In1), Cross Product/1
  norm/1(Out1) -> Square/1
  Direction Cosine Matrix to Quaternions/1 -> q_VNB/1
  Product1/1 -> Direction Cosine Matrix to Quaternions/1
  norm2/1(Out1) -> Divide3/2
  v_s/1 -> Divide3/1, norm2/1(v_s), Cross Product/2
  Divide3/1 -> Mux/1, Cross Product1/1
  Cross Product/1 -> Divide2/1, norm3/1(,), Divide4/1
  norm3/1(Out1) -> Divide4/2
  Divide4/1 -> Cross Product1/2, Mux/2
  Cross Product1/1 -> Mux/3
  mission_cmd/1 -> Subsystem/1(In1)
  Subsystem/1(Out3) -> Product/2, Product1/2
  Mux/1 -> Reshape/1
  Reshape/1 -> Product1/1
  Transpose2/1 -> w_VNB/1
  Divide2/1 -> Product/1

== system ADCS_v1/Subsystem1/Subsystem/default ==
  Action Port : ActionPort
  Constant : Constant  Value=[0; 0; 0]
  Constant1 : Constant  Value=[1 0 0 0]
  w_default : Outport
  q_default : Outport  Port=2
  wires:
  Constant1/1 -> q_default/1
  Constant/1 -> w_default/1

== system ADCS_v1/Subsystem2/Controller/Control Algorithms ==
  acs_mode : Inport
  CSS : Inport  Port=2
  omega : Inport  Port=3
  RW_omega : Inport  Port=4
  Camera feed : Inport  Port=5
  B : Inport  Port=6
  q_err : Inport  Port=7
  omega_err : Inport  Port=8
  DESAT : Subsystem  TreatAsAtomicUnit=on
  DETUMBLE1 : Subsystem  TreatAsAtomicUnit=on
  Merge : Merge
  RW Torque Commands : Subsystem
      settings: PortSchema="{\"entries\":[{\"content\":{\"sides\":[{\"content\":{\"connectorIds\":[\"In1\",\"In2\",\"In3\",\"In4\",\"In5\",\"In6\",\"In7\",\"In8\",\"In9\"]},\"type\":\"ConnectorPlacement.EquallySpacedRectSide\",\"uuid\":\"3d0ce77c-a0dd-4e63-bb58-aa259872b360\"},{\"content\":{\"connectorIds\":[\"Out1\"],\"side\":\"RIGHT\"},\"type\":\"ConnectorPlacement.EquallySpacedRectSide\",\"uuid\":\"c51ce6d0-00d2-499a-9be1-102c03c9909c\"},{\"content\":{\"connectorIds\":[\"In10\",\"In11\"],\"side\":\"TOP\"},\"type\":\"ConnectorPlacement.EquallySpacedRectSide\",\"uuid\":\"ed1e7bc4-2cca-4611-893f-1128994bf2d9\"}]},\"type\":\"ConnectorPlacement.EquallySpacedConnector\",\"uuid\":\"15c446ec-b512-4968-b865-507fd68d8b0b\"}],\"packageUris\":[\"http://schema.mathworks.com/mf0/Connector/R2020b\"],\"version\":\"1.0\"}"
  Switch Case1 : SwitchCase  CaseConditions={1,5}
  Switch Case2 : SwitchCase  CaseConditions={7}
  Switch Case3 : SwitchCase  CaseConditions={2,3,4,6,8,9}
  Thruster Torque commands : Subsystem
  omega_err1 : InportShadow  Port=8
  q_err1 : InportShadow  Port=7
  THR_tau : Outport
  MTQ_tau : Outport  Port=2
  RW_tau : Outport  Port=3
  wires:
  acs_mode/1 -> Switch Case1/1, Switch Case2/1, Switch Case3/1
  Switch Case3/7 -> RW Torque Commands/8(idle)
  Switch Case3/6 -> RW Torque Commands/7(safe)
  Switch Case3/5 -> RW Torque Commands/6(optical)
  Switch Case3/4 -> RW Torque Commands/5(spin)
  Switch Case3/3 -> RW Torque Commands/4(slew_slow)
  Switch Case3/2 -> RW Torque Commands/3(hold)
  Switch Case3/1 -> RW Torque Commands/2(point)
  Switch Case2/1 -> DESAT/Action
  Merge/1 -> MTQ_tau/1
  DESAT/1(tau_cmd) -> Merge/1
  Switch Case2/2 -> DETUMBLE1/Action
  DETUMBLE1/1(tau_cmd) -> Merge/2
  Switch Case1/3 -> Thruster Torque commands/3(default)
  Switch Case1/2 -> Thruster Torque commands/2(slew_fast)
  Switch Case1/1 -> Thruster Torque commands/1(detumble)
  q_err1/1 -> RW Torque Commands/11(q_err)
  omega_err1/1 -> RW Torque Commands/10(omega_err)
  q_err/1 -> Thruster Torque commands/5(q_err)
  omega_err/1 -> Thruster Torque commands/6(omega_err)
  omega/1 -> Thruster Torque commands/4(omega)
  Thruster Torque commands/1(tau_cmd) -> THR_tau/1
  CSS/1 -> RW Torque Commands/9(CSS)
  RW Torque Commands/1(tau_cmd) -> RW_tau/1
  B/1 -> DESAT/1(B)
  RW_omega/1 -> DESAT/2(RW_omega)
  Camera feed/1 -> RW Torque Commands/1(Camera feed)
